simulink model "sf_aircraft"  (R2025b)
settings: configuration reference "SharedConfig" (kept outside this file)
PreLoadFcn:
  | load_system('sf_aircraft_lib.slx');
  | load_system('sf_aircraft_controller.slx');
model workspace (MAT data in the model file):
  reset_cmd = 0
values from neighbouring files (symbols this model uses):
  ActuatorModeType : value not decoded    [sf_aircraft_dd.sldd]
undefined symbols (not defined in the file or in its folder): Left, noise_factor, Right
libraries: simulink x15, sf_aircraft_lib x4, SignalEditorBlockLib x1
(part 1 of 2)
settings Model: DataDictionary=sf_aircraft_dd.sldd  PacingRate=2  VariantFading=off  Creator=The MathWorks, Inc.  LastModifiedBy=The MathWorks, Inc.
settings ConfigSetRef: SourceName=SharedConfig

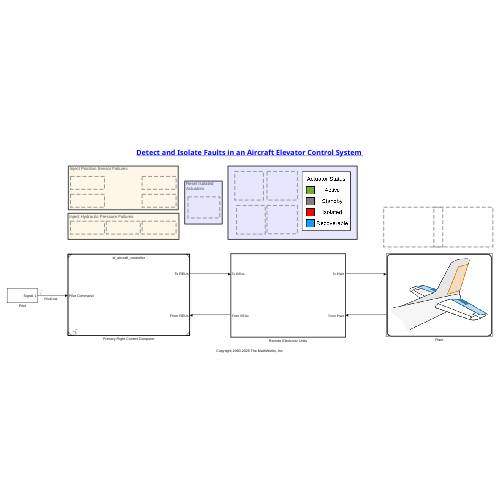
[thumbnail: Simulink's stored preview of the top-level diagram]
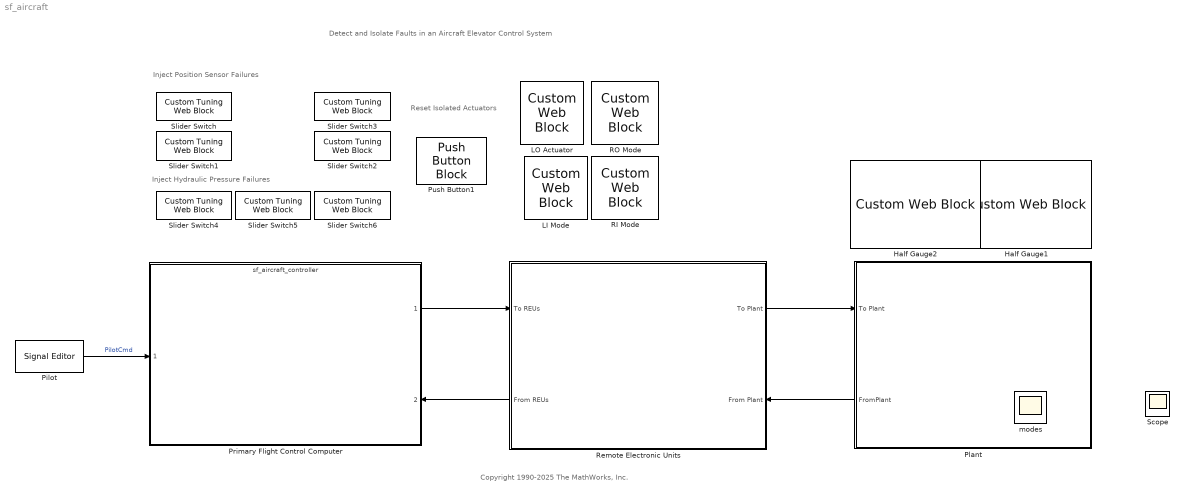
== system sf_aircraft ==
  note: Reset Isolated
      | Actuators
  note: Inject Hydraulic Pressure Failures
  note: Inject Position Sensor Failures
  note: Copyright 1990-2025 The MathWorks, Inc.
  note: Detect and Isolate Faults in an Aircraft Elevator Control System
  Half Gauge1 : CustomWebBlock  LabelPosition=Bottom  ShowInitialText=on  Configuration="{\"components\":[{\"name\":\"CircularScaleComponent\",\"settings\":{\"bounds\":{\"max\":1,\"min\":-1,\"tickInterval\":\"auto\"},\"direction\":\"cw\",\"flipLimits\":0,\"innerRadius\":0.75,\"internalTickHeightScaleFactor\":1,\"labelColor\":[255,255,200],\"labelFont\":{\"font\":\"Arial\",\"fontSize\":12},\"labelRadius\":0.528,\"labelTransparency\":1,\"minorTickHeightScaleFactor\":0.2,\"needleImage\":{\"size\":[200,50],\"src\":\"data:image\\/svg+xml;base64,PD94bWwgdmVyc2lvbj0iMS4wIiBlbmNvZGluZz0idXRmLTgiPz4KPCEtLSBHZW5lcmF0b3I6IEFkb2JlIElsbHVzdHJhdG9yIDI0LjEuMiwgU1ZHIEV4cG9ydCBQbHVnLUluIC4gU1ZHIFZlcnNpb246IDYuMDAgQnVpbGQgMCkgIC0tPgo8c3ZnIHZlcnNpb249IjEuMSIgaWQ9IkxheWVyXzEiIHhtbG5zPSJodHRwOi8vd3d3LnczLm9yZy8yMDAwL3N2ZyIgeG1sbnM6eGxpbms9Imh0dHA6Ly93d3cudzMub3JnLzE5OTkveGxpbmsiIHg9IjBweCIgeT0iMHB4IgoJIHZpZXdCb3g9IjAgMCAyMDAgNTAiIHN0eWxlPSJlbmFibGUtYmFja2dyb3VuZDpuZXcgMCAwIDIwMCA1MDsiIHhtbDpzcGFjZT0icHJlc2VydmUiPgo8c3R5bGUgdHlwZT0idGV4dC9jc3MiPgoJLnN0MHtmaWxsOiNFQzIxMjc7fQo8L3N0eWxlPgo8cGF0aCBjbGFzcz0ic3QwIiBkPSJNMTYyLjgsMTMuN0MxNjksNC40LDE4MS43LDEuOSwxOTEsOC4xczExLjgsMTguOSw1LjYsMjguMnMtMTguOSwxMS44LTI4LjIsNS42bDAsMAoJQzE1OS4xLDM1LjYsMTU2LjYsMjMsMTYyLjgsMTMuN0wxNjIuOCwxMy43eiBNMTY1LjgsMTUuOGMtNS4xLDcuNi0zLjEsMTcuOSw0LjYsMjNjNy42LDUuMSwxNy45LDMuMSwyMy00LjYKCWM1LjEtNy42LDMuMS0xNy45LTQuNi0yM2wwLDBDMTgxLjIsNi4yLDE3MC45LDguMiwxNjUuOCwxNS44eiIvPgo8cGF0aCBjbGFzcz0ic3QwIiBkPSJNMC40LDI1Ljl2LTMuM2wxNTktMi41Yy0wLjcsMi42LTAuNyw1LjIsMCw3LjhMMC40LDI1Ljl6Ii8+CjxjaXJjbGUgY2xhc3M9InN0MCIgY3g9IjE3OS42IiBjeT0iMjQiIHI9IjAuNyIvPgo8L3N2Zz4K\"},\"needleOffset\":[0.18464878250906522,0],\"needleOrientation\":-45,\"needleRotation\":180,\"needleSize\":{\"height\":0.11741692305346914,\"width\":0.46108337545091255},\"outerRadius\":0.9,\"position\":[-0.030336850649350648,0.09429505813953488,0.6517684108527132,1.0800527597402598],\"referencePoint\":\"auto\",\"scaleAngle\":120,\"scaleAngleOffset\":300,\"scaleColors\":[],\"scaleColorsSize\":0.2,\"scaleDirection\":\"CCW\",\"scalePosition\":[0,0,1,1],\"showLabels\":1,\"showMinorTicks\":1,\"showSpanLine\":1,\"showTicks\":1,\"tickColor\":[252,252,197],\"tickTransparency\":1,\"valueBarColor\":[0,0,0],\"valueBarPosition\":[0,0,1,1],\"valueBarSize\":0.2,\"valueBarTransparency\":1}},{\"name\":\"BackgroundImageComponent\",\"settings\":{\"image\":{\"size\":[0,0],\"src\":\"default\",\"srcOrientation\":\"Right\"},\"position\":[0,0,1,1],\"scaleMode\":\"0\"}},{\"name\":\"ForegroundImageComponent\",\"settings\":{\"image\":{\"size\":[0,0],\"src\":\"default\",\"srcOrientation\":[]},\"isForeground\":1,\"position\":[0,0,1,1],\"scaleMode\":\"0\"}}],\"derived\":{\"blockParameters\":{\"ForegroundColor\":[0.9882352941176471,0.9882352941176471,0.7725490196078432],\"Limits\":{\"Max\":1,\"Min\":-1,\"Ticks\":\"auto\"},\"ScaleColors\":[],\"ScaleDirection\":\"Counterclockwise\",\"ScaleMax\":1,\"ScaleMin\":-1,\"TickInterval\":\"auto\",\"fixedAspectRatio\":\"off\"}},\"settings\":{\"BindingType\":\"signal\",\"aspectRatio\":1.032258064516129,\"backgroundColor\":[0,0,0,\"1\"],\"backgroundOffset\":1,\"backgroundOpacity\":1,\"direction\":\"cw\",\"fixedAspectRatio\":\"off\",\"flipLimits\":0,\"orientation\":\"horizontal\",\"showBackgroundColor\":false,\"value\":0,\"version\":\"R2023a\"},\"type\":\"CircularGauge\"}"  CustomBackgroundColor="{\"color\":[0,0,0],\"show\":true}"
  Half Gauge2 : CustomWebBlock  LabelPosition=Bottom  ShowInitialText=on  Configuration="{\"components\":[{\"name\":\"CircularScaleComponent\",\"settings\":{\"bounds\":{\"max\":1,\"min\":-1,\"tickInterval\":\"auto\"},\"direction\":\"cw\",\"flipLimits\":0,\"innerRadius\":0.75,\"internalTickHeightScaleFactor\":1,\"labelColor\":[255,255,200],\"labelFont\":{\"font\":\"Arial\",\"fontSize\":12},\"labelRadius\":0.528,\"labelTransparency\":1,\"minorTickHeightScaleFactor\":0.2,\"needleImage\":{\"size\":[200,50],\"src\":\"data:image\\/svg+xml;base64,PD94bWwgdmVyc2lvbj0iMS4wIiBlbmNvZGluZz0idXRmLTgiPz4KPCEtLSBHZW5lcmF0b3I6IEFkb2JlIElsbHVzdHJhdG9yIDI0LjEuMiwgU1ZHIEV4cG9ydCBQbHVnLUluIC4gU1ZHIFZlcnNpb246IDYuMDAgQnVpbGQgMCkgIC0tPgo8c3ZnIHZlcnNpb249IjEuMSIgaWQ9IkxheWVyXzEiIHhtbG5zPSJodHRwOi8vd3d3LnczLm9yZy8yMDAwL3N2ZyIgeG1sbnM6eGxpbms9Imh0dHA6Ly93d3cudzMub3JnLzE5OTkveGxpbmsiIHg9IjBweCIgeT0iMHB4IgoJIHZpZXdCb3g9IjAgMCAyMDAgNTAiIHN0eWxlPSJlbmFibGUtYmFja2dyb3VuZDpuZXcgMCAwIDIwMCA1MDsiIHhtbDpzcGFjZT0icHJlc2VydmUiPgo8c3R5bGUgdHlwZT0idGV4dC9jc3MiPgoJLnN0MHtmaWxsOiNFQzIxMjc7fQo8L3N0eWxlPgo8cGF0aCBjbGFzcz0ic3QwIiBkPSJNMTYyLjgsMTMuN0MxNjksNC40LDE4MS43LDEuOSwxOTEsOC4xczExLjgsMTguOSw1LjYsMjguMnMtMTguOSwxMS44LTI4LjIsNS42bDAsMAoJQzE1OS4xLDM1LjYsMTU2LjYsMjMsMTYyLjgsMTMuN0wxNjIuOCwxMy43eiBNMTY1LjgsMTUuOGMtNS4xLDcuNi0zLjEsMTcuOSw0LjYsMjNjNy42LDUuMSwxNy45LDMuMSwyMy00LjYKCWM1LjEtNy42LDMuMS0xNy45LTQuNi0yM2wwLDBDMTgxLjIsNi4yLDE3MC45LDguMiwxNjUuOCwxNS44eiIvPgo8cGF0aCBjbGFzcz0ic3QwIiBkPSJNMC40LDI1Ljl2LTMuM2wxNTktMi41Yy0wLjcsMi42LTAuNyw1LjIsMCw3LjhMMC40LDI1Ljl6Ii8+CjxjaXJjbGUgY2xhc3M9InN0MCIgY3g9IjE3OS42IiBjeT0iMjQiIHI9IjAuNyIvPgo8L3N2Zz4K\"},\"needleOffset\":[0.18464878250906522,0],\"needleOrientation\":-45,\"needleRotation\":180,\"needleSize\":{\"height\":0.11741692305346914,\"width\":0.46108337545091255},\"outerRadius\":0.9,\"position\":[-0.012416294642857142,0.28617619493908153,0.6517806935332708,1.080078125],\"referencePoint\":\"auto\",\"scaleAngle\":120,\"scaleAngleOffset\":120,\"scaleColors\":[],\"scaleColorsSize\":0.2,\"scaleDirection\":\"CW\",\"scalePosition\":[0,0,1,1],\"showLabels\":1,\"showMinorTicks\":1,\"showSpanLine\":1,\"showTicks\":1,\"tickColor\":[252,252,197],\"tickTransparency\":1,\"valueBarColor\":[0,0,0],\"valueBarPosition\":[0,0,1,1],\"valueBarSize\":0.2,\"valueBarTransparency\":1}},{\"name\":\"BackgroundImageComponent\",\"settings\":{\"image\":{\"size\":[0,0],\"src\":\"default\",\"srcOrientation\":\"Right\"},\"position\":[0,0,1,1],\"scaleMode\":\"0\"}},{\"name\":\"ForegroundImageComponent\",\"settings\":{\"image\":{\"size\":[0,0],\"src\":\"default\",\"srcOrientation\":[]},\"isForeground\":1,\"position\":[0,0,1,1],\"scaleMode\":\"0\"}}],\"derived\":{\"blockParameters\":{\"ForegroundColor\":[0.9882352941176471,0.9882352941176471,0.7725490196078432],\"Limits\":{\"Max\":1,\"Min\":-1,\"Ticks\":\"auto\"},\"ScaleColors\":[],\"ScaleDirection\":\"Clockwise\",\"ScaleMax\":1,\"ScaleMin\":-1,\"TickInterval\":\"auto\",\"fixedAspectRatio\":\"on\"}},\"settings\":{\"BindingType\":\"signal\",\"aspectRatio\":1.032258064516129,\"backgroundColor\":[0,0,0,\"1\"],\"backgroundOffset\":1,\"backgroundOpacity\":1,\"direction\":\"cw\",\"fixedAspectRatio\":\"on\",\"flipLimits\":0,\"orientation\":\"horizontal\",\"showBackgroundColor\":false,\"value\":0,\"version\":\"R2023a\"},\"type\":\"CircularGauge\"}"  CustomBackgroundColor="{\"color\":[0,0,0],\"show\":true}"
  LI Mode : CustomWebBlock  LabelPosition=Bottom  ShowInitialText=on  Configuration="{\"components\":[{\"name\":\"BackgroundImageComponent\",\"settings\":{\"image\":{\"size\":[150,150],\"src\":\"data:image\\/svg+xml;base64,PHN2ZyB4bWxucz0iaHR0cDovL3d3dy53My5vcmcvMjAwMC9zdmciIHhtbG5zOnhsaW5rPSJodHRwOi8vd3d3LnczLm9yZy8xOTk5L3hsaW5rIiB2aWV3Qm94PSIwIDAgNTAwIDUwMCI+PGRlZnM+PHN0eWxlPi5he2ZpbGw6dXJsKCNhKTt9LmJ7ZmlsbDp1cmwoI2IpO30uY3tmaWxsOnVybCgjYyk7fTwvc3R5bGU+PHJhZGlhbEdyYWRpZW50IGlkPSJhIiBjeD0iMjgzLjg0IiBjeT0iLTQ2Ni4zNyIgcj0iMzc1Ljc1IiBncmFkaWVudFRyYW5zZm9ybT0ibWF0cml4KDEuMzksIDAsIDAsIC0xLjM5LCAtMTUzLjU2LCAtNjQ0LjA4KSIg ...(+2088 chars)\",\"srcOrientation\":\"Right\"},\"position\":[0,0,1,1],\"scaleMode\":\"0\"}},{\"name\":\"LampStateComponent\",\"settings\":{\"position\":[0,0,1,1],\"states\":[{\"icon\":{\"customSrc\":\"data:image\\/svg+xml;base64,PHN2ZyBpZD0iTGF5ZXJfMSIgZGF0YS1uYW1lPSJMYXllciAxIiB4bWxucz0iaHR0cDovL3d3dy53My5vcmcvMjAwMC9zdmciIHZpZXdCb3g9IjAgMCA0MTEgNDU4Ij48ZGVmcz48c3R5bGU+LmNscy0xe2ZpbGw6I2ZkZjhjMTt9LmNscy0ye2ZpbGw6I2ZlZTEwMDt9LmNscy0ze2ZpbGw6IzIzMWYyMDt9LmNscy00e2ZpbGw6I2EwOWY5Zjt9LmNscy00LC5jbHMtNSwuY2xzLTZ7c3Ryb2tlOiMyMzFmMjA7c3Ryb2tlLW1pdGVybGltaXQ6MTA7fS5jbHMtNXtmaWxsOiNmZmY7fS5jbHMtNntmaWxsOm5vbmU7fTwvc3R5bGU+PC9kZWZz ...(+5168 chars)\",\"id\":-1,\"srcOrientation\":\"Right\",\"type\":\"custom\"},\"iconScale\":0.8,\"metadata\":{},\"overlayType\":\"intersect\",\"shape\":{\"color\":[0.725,0,0],\"opacity\":1,\"position\":[0.1,0.1,0.8,0.8],\"type\":\"ellipse\"},\"value\":[]},{\"icon\":{\"customSrc\":\"data:image\\/svg+xml;base64,PHN2ZyBpZD0iTGF5ZXJfMSIgZGF0YS1uYW1lPSJMYXllciAxIiB4bWxucz0iaHR0cDovL3d3dy53My5vcmcvMjAwMC9zdmciIHZpZXdCb3g9IjAgMCA0MTEgNDU4Ij48ZGVmcz48c3R5bGU+LmNscy0xe2ZpbGw6I2ZkZjhjMTt9LmNscy0ye2ZpbGw6I2ZlZTEwMDt9LmNscy0ze2ZpbGw6IzIzMWYyMDt9LmNscy00e2ZpbGw6I2EwOWY5Zjt9LmNscy00LC5jbHMtNSwuY2xzLTZ7c3Ryb2tlOiMyMzFmMjA7c3Ryb2tlLW1pdGVybGltaXQ6MTA7fS5jbHMtNXtmaWxsOiNmZmY7fS5jbHMtNntmaWxsOm5vbmU7fTwvc3R5bGU+PC9kZWZz ...(+5168 chars)\",\"id\":-1,\"srcOrientation\":\"Right\",\"type\":\"custom\"},\"iconScale\":0.8,\"metadata\":{\"useDefaults\":{\"customIcon\":true,\"icon\":true,\"overlayType\":true,\"shape\":true,\"sizeAndPosition\":true}},\"overlayType\":\"intersect\",\"shape\":{\"color\":[0,0,0],\"opacity\":1,\"position\":[0.1,0.1,0.8,0.8],\"type\":\"ellipse\"},\"value\":\"0\"},{\"icon\":{\"customSrc\":\"data:image\\/svg+xml;base64,PHN2ZyBpZD0iTGF5ZXJfMSIgZGF0YS1uYW1lPSJMYXllciAxIiB4bWxucz0iaHR0cDovL3d3dy53My5vcmcvMjAwMC9zdmciIHZpZXdCb3g9IjAgMCA0MTEgNDU4Ij48ZGVmcz48c3R5bGU+LmNscy0xe2ZpbGw6I2ZkZjhjMTt9LmNscy0ye2ZpbGw6I2ZlZTEwMDt9LmNscy0ze2ZpbGw6IzIzMWYyMDt9LmNscy00e2ZpbGw6I2EwOWY5Zjt9LmNscy00LC5jbHMtNSwuY2xzLTZ7c3Ryb2tlOiMyMzFmMjA7c3Ryb2tlLW1pdGVybGltaXQ6MTA7fS5jbHMtNXtmaWxsOiNmZmY7fS5jbHMtNntmaWxsOm5vbmU7fTwvc3R5bGU+PC9kZWZz ...(+5168 chars)\",\"id\":-1,\"srcOrientation\":\"Right\",\"type\":\"custom\"},\"iconScale\":0.8,\"metadata\":{\"useDefaults\":{\"customIcon\":true,\"icon\":true,\"overlayType\":true,\"shape\":true,\"sizeAndPosition\":true}},\"overlayType\":\"intersect\",\"shape\":{\"color\":[0.4666666666666667,0.6745098039215687,0.18823529411764706],\"opacity\":1,\"position\":[0.1,0.1,0.8,0.8],\"type\":\"ellipse\"},\"value\":\"1\"},{\"icon\":{\"customSrc\":\"data:image\\/svg+xml;base64,PHN2ZyBpZD0iTGF5ZXJfMSIgZGF0YS1uYW1lPSJMYXllciAxIiB4bWxucz0iaHR0cDovL3d3dy53My5vcmcvMjAwMC9zdmciIHZpZXdCb3g9IjAgMCA0MTEgNDU4Ij48ZGVmcz48c3R5bGU+LmNscy0xe2ZpbGw6I2ZkZjhjMTt9LmNscy0ye2ZpbGw6I2ZlZTEwMDt9LmNscy0ze2ZpbGw6IzIzMWYyMDt9LmNscy00e2ZpbGw6I2EwOWY5Zjt9LmNscy00LC5jbHMtNSwuY2xzLTZ7c3Ryb2tlOiMyMzFmMjA7c3Ryb2tlLW1pdGVybGltaXQ6MTA7fS5jbHMtNXtmaWxsOiNmZmY7fS5jbHMtNntmaWxsOm5vbmU7fTwvc3R5bGU+PC9kZWZz ...(+5168 chars)\",\"id\":-1,\"srcOrientation\":\"Right\",\"type\":\"custom\"},\"iconScale\":0.8,\"metadata\":{\"useDefaults\":{\"customIcon\":true,\"icon\":true,\"overlayType\":true,\"shape\":true,\"sizeAndPosition\":true}},\"overlayType\":\"intersect\",\"shape\":{\"color\":[0.5019607843137255,0.5019607843137255,0.5019607843137255],\"opacity\":1,\"position\":[0.1,0.1,0.8,0.8],\"type\":\"ellipse\"},\"value\":\"2\"},{\"icon\":{\"customSrc\":\"data:image\\/svg+xml;base64,PHN2ZyBpZD0iTGF5ZXJfMSIgZGF0YS1uYW1lPSJMYXllciAxIiB4bWxucz0iaHR0cDovL3d3dy53My5vcmcvMjAwMC9zdmciIHZpZXdCb3g9IjAgMCA0MTEgNDU4Ij48ZGVmcz48c3R5bGU+LmNscy0xe2ZpbGw6I2ZkZjhjMTt9LmNscy0ye2ZpbGw6I2ZlZTEwMDt9LmNscy0ze2ZpbGw6IzIzMWYyMDt9LmNscy00e2ZpbGw6I2EwOWY5Zjt9LmNscy00LC5jbHMtNSwuY2xzLTZ7c3Ryb2tlOiMyMzFmMjA7c3Ryb2tlLW1pdGVybGltaXQ6MTA7fS5jbHMtNXtmaWxsOiNmZmY7fS5jbHMtNntmaWxsOm5vbmU7fTwvc3R5bGU+PC9kZWZz ...(+5168 chars)\",\"id\":-1,\"srcOrientation\":\"Right\",\"type\":\"custom\"},\"iconScale\":0.8,\"metadata\":{\"useDefaults\":{\"customIcon\":true,\"icon\":true,\"overlayType\":true,\"shape\":true,\"sizeAndPosition\":true}},\"overlayType\":\"intersect\",\"shape\":{\"color\":[1,0,0],\"opacity\":1,\"position\":[0.1,0.1,0.8,0.8],\"type\":\"ellipse\"},\"value\":\"3\"},{\"icon\":{\"customSrc\":\"data:image\\/svg+xml;base64,PHN2ZyBpZD0iTGF5ZXJfMSIgZGF0YS1uYW1lPSJMYXllciAxIiB4bWxucz0iaHR0cDovL3d3dy53My5vcmcvMjAwMC9zdmciIHZpZXdCb3g9IjAgMCA0MTEgNDU4Ij48ZGVmcz48c3R5bGU+LmNscy0xe2ZpbGw6I2ZkZjhjMTt9LmNscy0ye2ZpbGw6I2ZlZTEwMDt9LmNscy0ze2ZpbGw6IzIzMWYyMDt9LmNscy00e2ZpbGw6I2EwOWY5Zjt9LmNscy00LC5jbHMtNSwuY2xzLTZ7c3Ryb2tlOiMyMzFmMjA7c3Ryb2tlLW1pdGVybGltaXQ6MTA7fS5jbHMtNXtmaWxsOiNmZmY7fS5jbHMtNntmaWxsOm5vbmU7fTwvc3R5bGU+PC9kZWZz ...(+5168 chars)\",\"id\":-1,\"srcOrientation\":\"Right\",\"type\":\"custom\"},\"iconScale\":0.8,\"metadata\":{\"useDefaults\":{\"customIcon\":true,\"icon\":true,\"overlayType\":true,\"shape\":true,\"sizeAndPosition\":true}},\"overlayType\":\"intersect\",\"shape\":{\"color\":[0.07450980392156863,0.6235294117647059,1],\"opacity\":1,\"position\":[0.1,0.1,0.8,0.8],\"type\":\"ellipse\"},\"value\":\"4\"}],\"valueType\":\"discrete\"}},{\"name\":\"ForegroundImageComponent\",\"settings\":{\"image\":{\"size\":[150,150],\"src\":\"data:image\\/svg+xml;base64,PHN2ZyB4bWxucz0iaHR0cDovL3d3dy53My5vcmcvMjAwMC9zdmciIHhtbG5zOnhsaW5rPSJodHRwOi8vd3d3LnczLm9yZy8xOTk5L3hsaW5rIiB2aWV3Qm94PSIwIDAgNTAwIDUwMCI+PGRlZnM+PHN0eWxlPi5he2ZpbGw6dXJsKCNhKTt9PC9zdHlsZT48bGluZWFyR3JhZGllbnQgaWQ9ImEiIHgxPSIxNzMuMDUiIHkxPSItNjI3Ljc4IiB4Mj0iMTczLjA1IiB5Mj0iLTUyMi40MyIgZ3JhZGllbnRUcmFuc2Zvcm09Im1hdHJpeCgxLjI5LCAwLCAwLCAtMS4zMywgMjcuMTMsIC02MjguMzEpIiBncmFkaWVudFVuaXRzPSJ1c2VyU3BhY2VPblVzZSI+PHN0b3Agb2Zmc2V0PSIwIiBzdG9wLWNvbG9yPSIjZmZmIiBzdG9wLW9wYWNpdHk9IjAuMjUiLz48c3RvcCBvZmZzZXQ9IjEiIHN0b3AtY29sb3I9IiNmZmYiIHN0b3Atb3BhY2l0eT0iMCIvPjwvbGluZWFyR3JhZGllbnQ+PC9kZWZzPjxwYXRoIGNsYXNzPSJhIiBkPSJNNDI5LjMsMTkwLjY2QzQwMi40NSwxMTQuNTEsMzMyLjY3LDYwLjE3LDI1MC44NSw2MC4xN2MtODMuNDMsMC0xNTQuMjgsNTYuNDItMTc5Ljk1LDEzNSwxNS4zNCwzOSw4OC4xMSw3LDE3Ny4wNyw3QzM0MCwyMDIuMDgsNDE3LjI2LDIzNi40Niw0MjkuMywxOTAuNjZaIi8+PC9zdmc+\",\"srcOrientation\":\"Right\"},\"isForeground\":1,\"position\":[0,0,1,1],\"scaleMode\":\"0\"}}],\"derived\":{\"blockParameters\":{\"CustomIcon\":\"data:image\\/svg+xml;base64,PHN2ZyBpZD0iTGF5ZXJfMSIgZGF0YS1uYW1lPSJMYXllciAxIiB4bWxucz0iaHR0cDovL3d3dy53My5vcmcvMjAwMC9zdmciIHZpZXdCb3g9IjAgMCA0MTEgNDU4Ij48ZGVmcz48c3R5bGU+LmNscy0xe2ZpbGw6I2ZkZjhjMTt9LmNscy0ye2ZpbGw6I2ZlZTEwMDt9LmNscy0ze2ZpbGw6IzIzMWYyMDt9LmNscy00e2ZpbGw6I2EwOWY5Zjt9LmNscy00LC5jbHMtNSwuY2xzLTZ7c3Ryb2tlOiMyMzFmMjA7c3Ryb2tlLW1pdGVybGltaXQ6MTA7fS5jbHMtNXtmaWxsOiNmZmY7fS5jbHMtNntmaWxsOm5vbmU7fTwvc3R5bGU+PC9kZWZz ...(+5168 chars)\",\"DefaultColor\":[0.725,0,0],\"Icon\":\"Custom\",\"StateColors\":[{\"color\":[0,0,0],\"value\":\"0\"},{\"color\":[0.4666666666666667,0.6745098039215687,0.18823529411764706],\"value\":\"1\"},{\"color\":[0.5019607843137255,0.5019607843137255,0.5019607843137255],\"value\":\"2\"},{\"color\":[1,0,0],\"value\":\"3\"},{\"color\":[0.07450980392156863,0.6235294117647059,1],\"value\":\"4\"}],\"StateValueType\":\"discrete\",\"fixedAspectRatio\":\"off\"}},\"settings\":{\"BindingType\":\"signal\",\"aspectRatio\":1.032258064516129,\"backgroundColor\":[0,0,0],\"backgroundOffset\":0.14,\"backgroundOpacity\":1,\"blockOrientation\":\"Right\",\"fixedAspectRatio\":\"off\",\"showBackgroundColor\":false,\"value\":0,\"version\":\"R2023a\"},\"type\":\"Lamp\"}"
  "LO Actuator  " : CustomWebBlock  LabelPosition=Bottom  ShowInitialText=on  Configuration="{\"components\":[{\"name\":\"BackgroundImageComponent\",\"settings\":{\"image\":{\"size\":[150,150],\"src\":\"data:image\\/svg+xml;base64,PHN2ZyB4bWxucz0iaHR0cDovL3d3dy53My5vcmcvMjAwMC9zdmciIHhtbG5zOnhsaW5rPSJodHRwOi8vd3d3LnczLm9yZy8xOTk5L3hsaW5rIiB2aWV3Qm94PSIwIDAgNTAwIDUwMCI+PGRlZnM+PHN0eWxlPi5he2ZpbGw6dXJsKCNhKTt9LmJ7ZmlsbDp1cmwoI2IpO30uY3tmaWxsOnVybCgjYyk7fTwvc3R5bGU+PHJhZGlhbEdyYWRpZW50IGlkPSJhIiBjeD0iMjgzLjg0IiBjeT0iLTQ2Ni4zNyIgcj0iMzc1Ljc1IiBncmFkaWVudFRyYW5zZm9ybT0ibWF0cml4KDEuMzksIDAsIDAsIC0xLjM5LCAtMTUzLjU2LCAtNjQ0LjA4KSIg ...(+2088 chars)\",\"srcOrientation\":\"Right\"},\"position\":[0,0,1,1],\"scaleMode\":\"0\"}},{\"name\":\"LampStateComponent\",\"settings\":{\"position\":[0,0,1,1],\"states\":[{\"icon\":{\"customSrc\":\"data:image\\/svg+xml;base64,PHN2ZyBpZD0iTGF5ZXJfMSIgZGF0YS1uYW1lPSJMYXllciAxIiB4bWxucz0iaHR0cDovL3d3dy53My5vcmcvMjAwMC9zdmciIHZpZXdCb3g9IjAgMCA0MTEgNDU4Ij48ZGVmcz48c3R5bGU+LmNscy0xe2ZpbGw6I2ZkZjhjMTt9LmNscy0ye2ZpbGw6I2ZlZTEwMDt9LmNscy0ze2ZpbGw6IzIzMWYyMDt9LmNscy00e2ZpbGw6I2EwOWY5Zjt9LmNscy00LC5jbHMtNSwuY2xzLTZ7c3Ryb2tlOiMyMzFmMjA7c3Ryb2tlLW1pdGVybGltaXQ6MTA7fS5jbHMtNXtmaWxsOiNmZmY7fS5jbHMtNntmaWxsOm5vbmU7fTwvc3R5bGU+PC9kZWZz ...(+5168 chars)\",\"id\":-1,\"srcOrientation\":\"Right\",\"type\":\"custom\"},\"iconScale\":0.8,\"metadata\":{},\"overlayType\":\"intersect\",\"shape\":{\"color\":[0.725,0,0],\"opacity\":1,\"position\":[0.1,0.1,0.8,0.8],\"type\":\"ellipse\"},\"value\":[]},{\"icon\":{\"customSrc\":\"data:image\\/svg+xml;base64,PHN2ZyBpZD0iTGF5ZXJfMSIgZGF0YS1uYW1lPSJMYXllciAxIiB4bWxucz0iaHR0cDovL3d3dy53My5vcmcvMjAwMC9zdmciIHZpZXdCb3g9IjAgMCA0MTEgNDU4Ij48ZGVmcz48c3R5bGU+LmNscy0xe2ZpbGw6I2ZkZjhjMTt9LmNscy0ye2ZpbGw6I2ZlZTEwMDt9LmNscy0ze2ZpbGw6IzIzMWYyMDt9LmNscy00e2ZpbGw6I2EwOWY5Zjt9LmNscy00LC5jbHMtNSwuY2xzLTZ7c3Ryb2tlOiMyMzFmMjA7c3Ryb2tlLW1pdGVybGltaXQ6MTA7fS5jbHMtNXtmaWxsOiNmZmY7fS5jbHMtNntmaWxsOm5vbmU7fTwvc3R5bGU+PC9kZWZz ...(+5168 chars)\",\"id\":-1,\"srcOrientation\":\"Right\",\"type\":\"custom\"},\"iconScale\":0.8,\"metadata\":{\"useDefaults\":{\"customIcon\":true,\"icon\":true,\"overlayType\":true,\"shape\":true,\"sizeAndPosition\":true}},\"overlayType\":\"intersect\",\"shape\":{\"color\":[0,0,0],\"opacity\":1,\"position\":[0.1,0.1,0.8,0.8],\"type\":\"ellipse\"},\"value\":\"0\"},{\"icon\":{\"customSrc\":\"data:image\\/svg+xml;base64,PHN2ZyBpZD0iTGF5ZXJfMSIgZGF0YS1uYW1lPSJMYXllciAxIiB4bWxucz0iaHR0cDovL3d3dy53My5vcmcvMjAwMC9zdmciIHZpZXdCb3g9IjAgMCA0MTEgNDU4Ij48ZGVmcz48c3R5bGU+LmNscy0xe2ZpbGw6I2ZkZjhjMTt9LmNscy0ye2ZpbGw6I2ZlZTEwMDt9LmNscy0ze2ZpbGw6IzIzMWYyMDt9LmNscy00e2ZpbGw6I2EwOWY5Zjt9LmNscy00LC5jbHMtNSwuY2xzLTZ7c3Ryb2tlOiMyMzFmMjA7c3Ryb2tlLW1pdGVybGltaXQ6MTA7fS5jbHMtNXtmaWxsOiNmZmY7fS5jbHMtNntmaWxsOm5vbmU7fTwvc3R5bGU+PC9kZWZz ...(+5168 chars)\",\"id\":-1,\"srcOrientation\":\"Right\",\"type\":\"custom\"},\"iconScale\":0.8,\"metadata\":{\"useDefaults\":{\"customIcon\":true,\"icon\":true,\"overlayType\":true,\"shape\":true,\"sizeAndPosition\":true}},\"overlayType\":\"intersect\",\"shape\":{\"color\":[0.4666666666666667,0.6745098039215687,0.18823529411764706],\"opacity\":1,\"position\":[0.1,0.1,0.8,0.8],\"type\":\"ellipse\"},\"value\":\"1\"},{\"icon\":{\"customSrc\":\"data:image\\/svg+xml;base64,PHN2ZyBpZD0iTGF5ZXJfMSIgZGF0YS1uYW1lPSJMYXllciAxIiB4bWxucz0iaHR0cDovL3d3dy53My5vcmcvMjAwMC9zdmciIHZpZXdCb3g9IjAgMCA0MTEgNDU4Ij48ZGVmcz48c3R5bGU+LmNscy0xe2ZpbGw6I2ZkZjhjMTt9LmNscy0ye2ZpbGw6I2ZlZTEwMDt9LmNscy0ze2ZpbGw6IzIzMWYyMDt9LmNscy00e2ZpbGw6I2EwOWY5Zjt9LmNscy00LC5jbHMtNSwuY2xzLTZ7c3Ryb2tlOiMyMzFmMjA7c3Ryb2tlLW1pdGVybGltaXQ6MTA7fS5jbHMtNXtmaWxsOiNmZmY7fS5jbHMtNntmaWxsOm5vbmU7fTwvc3R5bGU+PC9kZWZz ...(+5168 chars)\",\"id\":-1,\"srcOrientation\":\"Right\",\"type\":\"custom\"},\"iconScale\":0.8,\"metadata\":{\"useDefaults\":{\"customIcon\":true,\"icon\":true,\"overlayType\":true,\"shape\":true,\"sizeAndPosition\":true}},\"overlayType\":\"intersect\",\"shape\":{\"color\":[0.5019607843137255,0.5019607843137255,0.5019607843137255],\"opacity\":1,\"position\":[0.1,0.1,0.8,0.8],\"type\":\"ellipse\"},\"value\":\"2\"},{\"icon\":{\"customSrc\":\"data:image\\/svg+xml;base64,PHN2ZyBpZD0iTGF5ZXJfMSIgZGF0YS1uYW1lPSJMYXllciAxIiB4bWxucz0iaHR0cDovL3d3dy53My5vcmcvMjAwMC9zdmciIHZpZXdCb3g9IjAgMCA0MTEgNDU4Ij48ZGVmcz48c3R5bGU+LmNscy0xe2ZpbGw6I2ZkZjhjMTt9LmNscy0ye2ZpbGw6I2ZlZTEwMDt9LmNscy0ze2ZpbGw6IzIzMWYyMDt9LmNscy00e2ZpbGw6I2EwOWY5Zjt9LmNscy00LC5jbHMtNSwuY2xzLTZ7c3Ryb2tlOiMyMzFmMjA7c3Ryb2tlLW1pdGVybGltaXQ6MTA7fS5jbHMtNXtmaWxsOiNmZmY7fS5jbHMtNntmaWxsOm5vbmU7fTwvc3R5bGU+PC9kZWZz ...(+5168 chars)\",\"id\":-1,\"srcOrientation\":\"Right\",\"type\":\"custom\"},\"iconScale\":0.8,\"metadata\":{\"useDefaults\":{\"customIcon\":true,\"icon\":true,\"overlayType\":true,\"shape\":true,\"sizeAndPosition\":true}},\"overlayType\":\"intersect\",\"shape\":{\"color\":[1,0,0],\"opacity\":1,\"position\":[0.1,0.1,0.8,0.8],\"type\":\"ellipse\"},\"value\":\"3\"},{\"icon\":{\"customSrc\":\"data:image\\/svg+xml;base64,PHN2ZyBpZD0iTGF5ZXJfMSIgZGF0YS1uYW1lPSJMYXllciAxIiB4bWxucz0iaHR0cDovL3d3dy53My5vcmcvMjAwMC9zdmciIHZpZXdCb3g9IjAgMCA0MTEgNDU4Ij48ZGVmcz48c3R5bGU+LmNscy0xe2ZpbGw6I2ZkZjhjMTt9LmNscy0ye2ZpbGw6I2ZlZTEwMDt9LmNscy0ze2ZpbGw6IzIzMWYyMDt9LmNscy00e2ZpbGw6I2EwOWY5Zjt9LmNscy00LC5jbHMtNSwuY2xzLTZ7c3Ryb2tlOiMyMzFmMjA7c3Ryb2tlLW1pdGVybGltaXQ6MTA7fS5jbHMtNXtmaWxsOiNmZmY7fS5jbHMtNntmaWxsOm5vbmU7fTwvc3R5bGU+PC9kZWZz ...(+5168 chars)\",\"id\":-1,\"srcOrientation\":\"Right\",\"type\":\"custom\"},\"iconScale\":0.8,\"metadata\":{\"useDefaults\":{\"customIcon\":true,\"icon\":true,\"overlayType\":true,\"shape\":true,\"sizeAndPosition\":true}},\"overlayType\":\"intersect\",\"shape\":{\"color\":[0.07450980392156863,0.6235294117647059,1],\"opacity\":1,\"position\":[0.1,0.1,0.8,0.8],\"type\":\"ellipse\"},\"value\":\"4\"}],\"valueType\":\"discrete\"}},{\"name\":\"ForegroundImageComponent\",\"settings\":{\"image\":{\"size\":[150,150],\"src\":\"data:image\\/svg+xml;base64,PHN2ZyB4bWxucz0iaHR0cDovL3d3dy53My5vcmcvMjAwMC9zdmciIHhtbG5zOnhsaW5rPSJodHRwOi8vd3d3LnczLm9yZy8xOTk5L3hsaW5rIiB2aWV3Qm94PSIwIDAgNTAwIDUwMCI+PGRlZnM+PHN0eWxlPi5he2ZpbGw6dXJsKCNhKTt9PC9zdHlsZT48bGluZWFyR3JhZGllbnQgaWQ9ImEiIHgxPSIxNzMuMDUiIHkxPSItNjI3Ljc4IiB4Mj0iMTczLjA1IiB5Mj0iLTUyMi40MyIgZ3JhZGllbnRUcmFuc2Zvcm09Im1hdHJpeCgxLjI5LCAwLCAwLCAtMS4zMywgMjcuMTMsIC02MjguMzEpIiBncmFkaWVudFVuaXRzPSJ1c2VyU3BhY2VPblVzZSI+PHN0b3Agb2Zmc2V0PSIwIiBzdG9wLWNvbG9yPSIjZmZmIiBzdG9wLW9wYWNpdHk9IjAuMjUiLz48c3RvcCBvZmZzZXQ9IjEiIHN0b3AtY29sb3I9IiNmZmYiIHN0b3Atb3BhY2l0eT0iMCIvPjwvbGluZWFyR3JhZGllbnQ+PC9kZWZzPjxwYXRoIGNsYXNzPSJhIiBkPSJNNDI5LjMsMTkwLjY2QzQwMi40NSwxMTQuNTEsMzMyLjY3LDYwLjE3LDI1MC44NSw2MC4xN2MtODMuNDMsMC0xNTQuMjgsNTYuNDItMTc5Ljk1LDEzNSwxNS4zNCwzOSw4OC4xMSw3LDE3Ny4wNyw3QzM0MCwyMDIuMDgsNDE3LjI2LDIzNi40Niw0MjkuMywxOTAuNjZaIi8+PC9zdmc+\",\"srcOrientation\":\"Right\"},\"isForeground\":1,\"position\":[0,0,1,1],\"scaleMode\":\"0\"}}],\"derived\":{\"blockParameters\":{\"CustomIcon\":\"data:image\\/svg+xml;base64,PHN2ZyBpZD0iTGF5ZXJfMSIgZGF0YS1uYW1lPSJMYXllciAxIiB4bWxucz0iaHR0cDovL3d3dy53My5vcmcvMjAwMC9zdmciIHZpZXdCb3g9IjAgMCA0MTEgNDU4Ij48ZGVmcz48c3R5bGU+LmNscy0xe2ZpbGw6I2ZkZjhjMTt9LmNscy0ye2ZpbGw6I2ZlZTEwMDt9LmNscy0ze2ZpbGw6IzIzMWYyMDt9LmNscy00e2ZpbGw6I2EwOWY5Zjt9LmNscy00LC5jbHMtNSwuY2xzLTZ7c3Ryb2tlOiMyMzFmMjA7c3Ryb2tlLW1pdGVybGltaXQ6MTA7fS5jbHMtNXtmaWxsOiNmZmY7fS5jbHMtNntmaWxsOm5vbmU7fTwvc3R5bGU+PC9kZWZz ...(+5168 chars)\",\"DefaultColor\":[0.725,0,0],\"Icon\":\"Custom\",\"StateColors\":[{\"color\":[0,0,0],\"value\":\"0\"},{\"color\":[0.4666666666666667,0.6745098039215687,0.18823529411764706],\"value\":\"1\"},{\"color\":[0.5019607843137255,0.5019607843137255,0.5019607843137255],\"value\":\"2\"},{\"color\":[1,0,0],\"value\":\"3\"},{\"color\":[0.07450980392156863,0.6235294117647059,1],\"value\":\"4\"}],\"StateValueType\":\"discrete\",\"fixedAspectRatio\":\"off\"}},\"settings\":{\"BindingType\":\"signal\",\"aspectRatio\":1.032258064516129,\"backgroundColor\":[0,0,0],\"backgroundOffset\":0.14,\"backgroundOpacity\":1,\"blockOrientation\":\"Right\",\"fixedAspectRatio\":\"off\",\"showBackgroundColor\":false,\"value\":0,\"version\":\"R2023a\"},\"type\":\"Lamp\"}"
  Pilot : SignalEditorBlockLib/Signal Editor  FileName=simplepilot.mat  ActiveScenario=Takeoff  ActiveSignal=Signal 1  IsBus=off  OutputBusObjectStr=Bus: BusObject  SampleTime=.1  Interpolate=off  ZeroCross=off  OutputAfterFinalValue=Setting to zero  Unit=inherit  PreserveSignalName=on  ApplySigPropsToAllScenarios=on  ApplySigPropsToAllSignals=off  SignalPropertySource=Dialog parameters
  Plant : Subsystem
      settings: PortSchema="{\"entries\":[{\"content\":{\"sides\":[{\"content\":{\"connectorIds\":[\"In1\",\"Out1\"]},\"type\":\"ConnectorPlacement.EquallySpacedRectSide\",\"uuid\":\"38682bff-efe9-4f74-b563-7d17327409bc\"},{\"content\":{\"side\":\"RIGHT\"},\"type\":\"ConnectorPlacement.EquallySpacedRectSide\",\"uuid\":\"9b27296a-7a15-43c2-9a49-3690713ba5ee\"},{\"content\":{\"side\":\"TOP\"},\"type\":\"ConnectorPlacement.EquallySpacedRectSide\",\"uuid\":\"df0d1eaf-2d63-4586-9b70-ab9eb3cbba48\"}]},\"type\":\"ConnectorPlacement.EquallySpacedConnector\",\"uuid\":\"3720bb81-e23a-4071-aa80-868b0be59702\"}],\"packageUris\":[\"http://schema.mathworks.com/mf0/Connector/R2020b\"],\"version\":\"1.0\"}"
      mask Display: image('aircraft-elevator.png');
  Primary Flight Control Computer : ModelReference  ModelNameDialog=sf_aircraft_controller  SimulationMode=Normal  ModelReferenceVersion=2.13
      settings: PortSchema="{\"entries\":[{\"content\":{\"sides\":[{\"content\":{\"connectorIds\":[\"In1\"]},\"type\":\"ConnectorPlacement.EquallySpacedRectSide\",\"uuid\":\"4aa03f90-93a0-4c7f-a3cd-6daab17b3951\"},{\"content\":{\"connectorIds\":[\"Out1\",\"In2\"],\"side\":\"RIGHT\"},\"type\":\"ConnectorPlacement.EquallySpacedRectSide\",\"uuid\":\"3b750c9f-37e0-4721-beac-0d825a86c64b\"},{\"content\":{\"side\":\"TOP\"},\"type\":\"ConnectorPlacement.EquallySpacedRectSide\",\"uuid\":\"845b3102-9354-404f-9f20-8ca6a930b73c\"}]},\"type\":\"ConnectorPlacement.EquallySpacedConnector\",\"uuid\":\"f07501ae-eb53-443d-bbea-7ab38e30640c\"}],\"packageUris\":[\"http://schema.mathworks.com/mf0/Connector/R2020b\"],\"version\":\"1.0\"}"
  Push Button1 : PushButtonBlock  Icon=Custom  CustomIcon=data:image/png;base64,iVBORw0KGgoAAAANSUhEUgAABQAAAAQyCAYAAAD3IVLlAAVlcklEQVR42uyYP2gUQRSHL/FSCNrYWIhgYSUIgmCZYKWFjUUqRXBnNrszk7vNxuSSS3ONFgpaiAiKXiGBoEK0sFAMiohCCsV/CCrEIoUBISQ7s94lJvf87XJwsTaN4X3wMe+9mTePZbotMAzDMAzDbEWoUOiq1WrdlNnfvy0TcZFqfcV7WUzUVdgknvfh3lFv54IQuxtBsC8pBQdSJQ8n2ut1oTyWGHnSKnE6NdI45Y84JaqJljUbyvNWy4tOySuJFtdSLW8gr2N/Et6F08gfwSfOiGfIX1olZ+Fb9HxE/sVqMYd13mm5gHgRscWsJnpacC2LocPeEnp+ovcH4nn4HfWv6PuMng+o ...(+471212 chars)  IconAlignment=Top  IconOnColor=[0.0, 0.39215686274509803, 0.0]  IconOffColor=[0.0, 1.0, 0.0]  OffValue=0.000000
  RI Mode : CustomWebBlock  LabelPosition=Bottom  ShowInitialText=on  Configuration="{\"components\":[{\"name\":\"BackgroundImageComponent\",\"settings\":{\"image\":{\"size\":[150,150],\"src\":\"data:image\\/svg+xml;base64,PHN2ZyB4bWxucz0iaHR0cDovL3d3dy53My5vcmcvMjAwMC9zdmciIHhtbG5zOnhsaW5rPSJodHRwOi8vd3d3LnczLm9yZy8xOTk5L3hsaW5rIiB2aWV3Qm94PSIwIDAgNTAwIDUwMCI+PGRlZnM+PHN0eWxlPi5he2ZpbGw6dXJsKCNhKTt9LmJ7ZmlsbDp1cmwoI2IpO30uY3tmaWxsOnVybCgjYyk7fTwvc3R5bGU+PHJhZGlhbEdyYWRpZW50IGlkPSJhIiBjeD0iMjgzLjg0IiBjeT0iLTQ2Ni4zNyIgcj0iMzc1Ljc1IiBncmFkaWVudFRyYW5zZm9ybT0ibWF0cml4KDEuMzksIDAsIDAsIC0xLjM5LCAtMTUzLjU2LCAtNjQ0LjA4KSIg ...(+2088 chars)\",\"srcOrientation\":\"Right\"},\"position\":[0,0,1,1],\"scaleMode\":\"0\"}},{\"name\":\"LampStateComponent\",\"settings\":{\"position\":[0,0,1,1],\"states\":[{\"icon\":{\"customSrc\":\"data:image\\/svg+xml;base64,PHN2ZyBpZD0iTGF5ZXJfMSIgZGF0YS1uYW1lPSJMYXllciAxIiB4bWxucz0iaHR0cDovL3d3dy53My5vcmcvMjAwMC9zdmciIHZpZXdCb3g9IjAgMCA0MTEgNDU4Ij48ZGVmcz48c3R5bGU+LmNscy0xe2ZpbGw6I2ZkZjhjMTt9LmNscy0ye2ZpbGw6I2ZlZTEwMDt9LmNscy0ze2ZpbGw6IzIzMWYyMDt9LmNscy00e2ZpbGw6I2EwOWY5Zjt9LmNscy00LC5jbHMtNSwuY2xzLTZ7c3Ryb2tlOiMyMzFmMjA7c3Ryb2tlLW1pdGVybGltaXQ6MTA7fS5jbHMtNXtmaWxsOiNmZmY7fS5jbHMtNntmaWxsOm5vbmU7fTwvc3R5bGU+PC9kZWZz ...(+5168 chars)\",\"id\":-1,\"srcOrientation\":\"Right\",\"type\":\"custom\"},\"iconScale\":0.8,\"metadata\":{},\"overlayType\":\"intersect\",\"shape\":{\"color\":[0.725,0,0],\"opacity\":1,\"position\":[0.1,0.1,0.8,0.8],\"type\":\"ellipse\"},\"value\":[]},{\"icon\":{\"customSrc\":\"data:image\\/svg+xml;base64,PHN2ZyBpZD0iTGF5ZXJfMSIgZGF0YS1uYW1lPSJMYXllciAxIiB4bWxucz0iaHR0cDovL3d3dy53My5vcmcvMjAwMC9zdmciIHZpZXdCb3g9IjAgMCA0MTEgNDU4Ij48ZGVmcz48c3R5bGU+LmNscy0xe2ZpbGw6I2ZkZjhjMTt9LmNscy0ye2ZpbGw6I2ZlZTEwMDt9LmNscy0ze2ZpbGw6IzIzMWYyMDt9LmNscy00e2ZpbGw6I2EwOWY5Zjt9LmNscy00LC5jbHMtNSwuY2xzLTZ7c3Ryb2tlOiMyMzFmMjA7c3Ryb2tlLW1pdGVybGltaXQ6MTA7fS5jbHMtNXtmaWxsOiNmZmY7fS5jbHMtNntmaWxsOm5vbmU7fTwvc3R5bGU+PC9kZWZz ...(+5168 chars)\",\"id\":-1,\"srcOrientation\":\"Right\",\"type\":\"custom\"},\"iconScale\":0.8,\"metadata\":{\"useDefaults\":{\"customIcon\":true,\"icon\":true,\"overlayType\":true,\"shape\":true,\"sizeAndPosition\":true}},\"overlayType\":\"intersect\",\"shape\":{\"color\":[0,0,0],\"opacity\":1,\"position\":[0.1,0.1,0.8,0.8],\"type\":\"ellipse\"},\"value\":\"0\"},{\"icon\":{\"customSrc\":\"data:image\\/svg+xml;base64,PHN2ZyBpZD0iTGF5ZXJfMSIgZGF0YS1uYW1lPSJMYXllciAxIiB4bWxucz0iaHR0cDovL3d3dy53My5vcmcvMjAwMC9zdmciIHZpZXdCb3g9IjAgMCA0MTEgNDU4Ij48ZGVmcz48c3R5bGU+LmNscy0xe2ZpbGw6I2ZkZjhjMTt9LmNscy0ye2ZpbGw6I2ZlZTEwMDt9LmNscy0ze2ZpbGw6IzIzMWYyMDt9LmNscy00e2ZpbGw6I2EwOWY5Zjt9LmNscy00LC5jbHMtNSwuY2xzLTZ7c3Ryb2tlOiMyMzFmMjA7c3Ryb2tlLW1pdGVybGltaXQ6MTA7fS5jbHMtNXtmaWxsOiNmZmY7fS5jbHMtNntmaWxsOm5vbmU7fTwvc3R5bGU+PC9kZWZz ...(+5168 chars)\",\"id\":-1,\"srcOrientation\":\"Right\",\"type\":\"custom\"},\"iconScale\":0.8,\"metadata\":{\"useDefaults\":{\"customIcon\":true,\"icon\":true,\"overlayType\":true,\"shape\":true,\"sizeAndPosition\":true}},\"overlayType\":\"intersect\",\"shape\":{\"color\":[0.4666666666666667,0.6745098039215687,0.18823529411764706],\"opacity\":1,\"position\":[0.1,0.1,0.8,0.8],\"type\":\"ellipse\"},\"value\":\"1\"},{\"icon\":{\"customSrc\":\"data:image\\/svg+xml;base64,PHN2ZyBpZD0iTGF5ZXJfMSIgZGF0YS1uYW1lPSJMYXllciAxIiB4bWxucz0iaHR0cDovL3d3dy53My5vcmcvMjAwMC9zdmciIHZpZXdCb3g9IjAgMCA0MTEgNDU4Ij48ZGVmcz48c3R5bGU+LmNscy0xe2ZpbGw6I2ZkZjhjMTt9LmNscy0ye2ZpbGw6I2ZlZTEwMDt9LmNscy0ze2ZpbGw6IzIzMWYyMDt9LmNscy00e2ZpbGw6I2EwOWY5Zjt9LmNscy00LC5jbHMtNSwuY2xzLTZ7c3Ryb2tlOiMyMzFmMjA7c3Ryb2tlLW1pdGVybGltaXQ6MTA7fS5jbHMtNXtmaWxsOiNmZmY7fS5jbHMtNntmaWxsOm5vbmU7fTwvc3R5bGU+PC9kZWZz ...(+5168 chars)\",\"id\":-1,\"srcOrientation\":\"Right\",\"type\":\"custom\"},\"iconScale\":0.8,\"metadata\":{\"useDefaults\":{\"customIcon\":true,\"icon\":true,\"overlayType\":true,\"shape\":true,\"sizeAndPosition\":true}},\"overlayType\":\"intersect\",\"shape\":{\"color\":[0.5019607843137255,0.5019607843137255,0.5019607843137255],\"opacity\":1,\"position\":[0.1,0.1,0.8,0.8],\"type\":\"ellipse\"},\"value\":\"2\"},{\"icon\":{\"customSrc\":\"data:image\\/svg+xml;base64,PHN2ZyBpZD0iTGF5ZXJfMSIgZGF0YS1uYW1lPSJMYXllciAxIiB4bWxucz0iaHR0cDovL3d3dy53My5vcmcvMjAwMC9zdmciIHZpZXdCb3g9IjAgMCA0MTEgNDU4Ij48ZGVmcz48c3R5bGU+LmNscy0xe2ZpbGw6I2ZkZjhjMTt9LmNscy0ye2ZpbGw6I2ZlZTEwMDt9LmNscy0ze2ZpbGw6IzIzMWYyMDt9LmNscy00e2ZpbGw6I2EwOWY5Zjt9LmNscy00LC5jbHMtNSwuY2xzLTZ7c3Ryb2tlOiMyMzFmMjA7c3Ryb2tlLW1pdGVybGltaXQ6MTA7fS5jbHMtNXtmaWxsOiNmZmY7fS5jbHMtNntmaWxsOm5vbmU7fTwvc3R5bGU+PC9kZWZz ...(+5168 chars)\",\"id\":-1,\"srcOrientation\":\"Right\",\"type\":\"custom\"},\"iconScale\":0.8,\"metadata\":{\"useDefaults\":{\"customIcon\":true,\"icon\":true,\"overlayType\":true,\"shape\":true,\"sizeAndPosition\":true}},\"overlayType\":\"intersect\",\"shape\":{\"color\":[1,0,0],\"opacity\":1,\"position\":[0.1,0.1,0.8,0.8],\"type\":\"ellipse\"},\"value\":\"3\"},{\"icon\":{\"customSrc\":\"data:image\\/svg+xml;base64,PHN2ZyBpZD0iTGF5ZXJfMSIgZGF0YS1uYW1lPSJMYXllciAxIiB4bWxucz0iaHR0cDovL3d3dy53My5vcmcvMjAwMC9zdmciIHZpZXdCb3g9IjAgMCA0MTEgNDU4Ij48ZGVmcz48c3R5bGU+LmNscy0xe2ZpbGw6I2ZkZjhjMTt9LmNscy0ye2ZpbGw6I2ZlZTEwMDt9LmNscy0ze2ZpbGw6IzIzMWYyMDt9LmNscy00e2ZpbGw6I2EwOWY5Zjt9LmNscy00LC5jbHMtNSwuY2xzLTZ7c3Ryb2tlOiMyMzFmMjA7c3Ryb2tlLW1pdGVybGltaXQ6MTA7fS5jbHMtNXtmaWxsOiNmZmY7fS5jbHMtNntmaWxsOm5vbmU7fTwvc3R5bGU+PC9kZWZz ...(+5168 chars)\",\"id\":-1,\"srcOrientation\":\"Right\",\"type\":\"custom\"},\"iconScale\":0.8,\"metadata\":{\"useDefaults\":{\"customIcon\":true,\"icon\":true,\"overlayType\":true,\"shape\":true,\"sizeAndPosition\":true}},\"overlayType\":\"intersect\",\"shape\":{\"color\":[0.07450980392156863,0.6235294117647059,1],\"opacity\":1,\"position\":[0.1,0.1,0.8,0.8],\"type\":\"ellipse\"},\"value\":\"4\"}],\"valueType\":\"discrete\"}},{\"name\":\"ForegroundImageComponent\",\"settings\":{\"image\":{\"size\":[150,150],\"src\":\"data:image\\/svg+xml;base64,PHN2ZyB4bWxucz0iaHR0cDovL3d3dy53My5vcmcvMjAwMC9zdmciIHhtbG5zOnhsaW5rPSJodHRwOi8vd3d3LnczLm9yZy8xOTk5L3hsaW5rIiB2aWV3Qm94PSIwIDAgNTAwIDUwMCI+PGRlZnM+PHN0eWxlPi5he2ZpbGw6dXJsKCNhKTt9PC9zdHlsZT48bGluZWFyR3JhZGllbnQgaWQ9ImEiIHgxPSIxNzMuMDUiIHkxPSItNjI3Ljc4IiB4Mj0iMTczLjA1IiB5Mj0iLTUyMi40MyIgZ3JhZGllbnRUcmFuc2Zvcm09Im1hdHJpeCgxLjI5LCAwLCAwLCAtMS4zMywgMjcuMTMsIC02MjguMzEpIiBncmFkaWVudFVuaXRzPSJ1c2VyU3BhY2VPblVzZSI+PHN0b3Agb2Zmc2V0PSIwIiBzdG9wLWNvbG9yPSIjZmZmIiBzdG9wLW9wYWNpdHk9IjAuMjUiLz48c3RvcCBvZmZzZXQ9IjEiIHN0b3AtY29sb3I9IiNmZmYiIHN0b3Atb3BhY2l0eT0iMCIvPjwvbGluZWFyR3JhZGllbnQ+PC9kZWZzPjxwYXRoIGNsYXNzPSJhIiBkPSJNNDI5LjMsMTkwLjY2QzQwMi40NSwxMTQuNTEsMzMyLjY3LDYwLjE3LDI1MC44NSw2MC4xN2MtODMuNDMsMC0xNTQuMjgsNTYuNDItMTc5Ljk1LDEzNSwxNS4zNCwzOSw4OC4xMSw3LDE3Ny4wNyw3QzM0MCwyMDIuMDgsNDE3LjI2LDIzNi40Niw0MjkuMywxOTAuNjZaIi8+PC9zdmc+\",\"srcOrientation\":\"Right\"},\"isForeground\":1,\"position\":[0,0,1,1],\"scaleMode\":\"0\"}}],\"derived\":{\"blockParameters\":{\"CustomIcon\":\"data:image\\/svg+xml;base64,PHN2ZyBpZD0iTGF5ZXJfMSIgZGF0YS1uYW1lPSJMYXllciAxIiB4bWxucz0iaHR0cDovL3d3dy53My5vcmcvMjAwMC9zdmciIHZpZXdCb3g9IjAgMCA0MTEgNDU4Ij48ZGVmcz48c3R5bGU+LmNscy0xe2ZpbGw6I2ZkZjhjMTt9LmNscy0ye2ZpbGw6I2ZlZTEwMDt9LmNscy0ze2ZpbGw6IzIzMWYyMDt9LmNscy00e2ZpbGw6I2EwOWY5Zjt9LmNscy00LC5jbHMtNSwuY2xzLTZ7c3Ryb2tlOiMyMzFmMjA7c3Ryb2tlLW1pdGVybGltaXQ6MTA7fS5jbHMtNXtmaWxsOiNmZmY7fS5jbHMtNntmaWxsOm5vbmU7fTwvc3R5bGU+PC9kZWZz ...(+5168 chars)\",\"DefaultColor\":[0.725,0,0],\"Icon\":\"Custom\",\"StateColors\":[{\"color\":[0,0,0],\"value\":\"0\"},{\"color\":[0.4666666666666667,0.6745098039215687,0.18823529411764706],\"value\":\"1\"},{\"color\":[0.5019607843137255,0.5019607843137255,0.5019607843137255],\"value\":\"2\"},{\"color\":[1,0,0],\"value\":\"3\"},{\"color\":[0.07450980392156863,0.6235294117647059,1],\"value\":\"4\"}],\"StateValueType\":\"discrete\",\"fixedAspectRatio\":\"off\"}},\"settings\":{\"BindingType\":\"signal\",\"aspectRatio\":1.032258064516129,\"backgroundColor\":[0,0,0],\"backgroundOffset\":0.14,\"backgroundOpacity\":1,\"blockOrientation\":\"Right\",\"fixedAspectRatio\":\"off\",\"showBackgroundColor\":false,\"value\":0,\"version\":\"R2023a\"},\"type\":\"Lamp\"}"
  RO Mode : CustomWebBlock  LabelPosition=Bottom  ShowInitialText=on  Configuration="{\"components\":[{\"name\":\"BackgroundImageComponent\",\"settings\":{\"image\":{\"size\":[150,150],\"src\":\"data:image\\/svg+xml;base64,PHN2ZyB4bWxucz0iaHR0cDovL3d3dy53My5vcmcvMjAwMC9zdmciIHhtbG5zOnhsaW5rPSJodHRwOi8vd3d3LnczLm9yZy8xOTk5L3hsaW5rIiB2aWV3Qm94PSIwIDAgNTAwIDUwMCI+PGRlZnM+PHN0eWxlPi5he2ZpbGw6dXJsKCNhKTt9LmJ7ZmlsbDp1cmwoI2IpO30uY3tmaWxsOnVybCgjYyk7fTwvc3R5bGU+PHJhZGlhbEdyYWRpZW50IGlkPSJhIiBjeD0iMjgzLjg0IiBjeT0iLTQ2Ni4zNyIgcj0iMzc1Ljc1IiBncmFkaWVudFRyYW5zZm9ybT0ibWF0cml4KDEuMzksIDAsIDAsIC0xLjM5LCAtMTUzLjU2LCAtNjQ0LjA4KSIg ...(+2088 chars)\",\"srcOrientation\":\"Right\"},\"position\":[0,0,1,1],\"scaleMode\":\"0\"}},{\"name\":\"LampStateComponent\",\"settings\":{\"position\":[0,0,1,1],\"states\":[{\"icon\":{\"customSrc\":\"data:image\\/svg+xml;base64,PHN2ZyBpZD0iTGF5ZXJfMSIgZGF0YS1uYW1lPSJMYXllciAxIiB4bWxucz0iaHR0cDovL3d3dy53My5vcmcvMjAwMC9zdmciIHZpZXdCb3g9IjAgMCA0MTEgNDU4Ij48ZGVmcz48c3R5bGU+LmNscy0xe2ZpbGw6I2ZkZjhjMTt9LmNscy0ye2ZpbGw6I2ZlZTEwMDt9LmNscy0ze2ZpbGw6IzIzMWYyMDt9LmNscy00e2ZpbGw6I2EwOWY5Zjt9LmNscy00LC5jbHMtNSwuY2xzLTZ7c3Ryb2tlOiMyMzFmMjA7c3Ryb2tlLW1pdGVybGltaXQ6MTA7fS5jbHMtNXtmaWxsOiNmZmY7fS5jbHMtNntmaWxsOm5vbmU7fTwvc3R5bGU+PC9kZWZz ...(+5168 chars)\",\"id\":-1,\"srcOrientation\":\"Right\",\"type\":\"custom\"},\"iconScale\":0.8,\"metadata\":{},\"overlayType\":\"intersect\",\"shape\":{\"color\":[0.725,0,0],\"opacity\":1,\"position\":[0.1,0.1,0.8,0.8],\"type\":\"ellipse\"},\"value\":[]},{\"icon\":{\"customSrc\":\"data:image\\/svg+xml;base64,PHN2ZyBpZD0iTGF5ZXJfMSIgZGF0YS1uYW1lPSJMYXllciAxIiB4bWxucz0iaHR0cDovL3d3dy53My5vcmcvMjAwMC9zdmciIHZpZXdCb3g9IjAgMCA0MTEgNDU4Ij48ZGVmcz48c3R5bGU+LmNscy0xe2ZpbGw6I2ZkZjhjMTt9LmNscy0ye2ZpbGw6I2ZlZTEwMDt9LmNscy0ze2ZpbGw6IzIzMWYyMDt9LmNscy00e2ZpbGw6I2EwOWY5Zjt9LmNscy00LC5jbHMtNSwuY2xzLTZ7c3Ryb2tlOiMyMzFmMjA7c3Ryb2tlLW1pdGVybGltaXQ6MTA7fS5jbHMtNXtmaWxsOiNmZmY7fS5jbHMtNntmaWxsOm5vbmU7fTwvc3R5bGU+PC9kZWZz ...(+5168 chars)\",\"id\":-1,\"srcOrientation\":\"Right\",\"type\":\"custom\"},\"iconScale\":0.8,\"metadata\":{\"useDefaults\":{\"customIcon\":true,\"icon\":true,\"overlayType\":true,\"shape\":true,\"sizeAndPosition\":true}},\"overlayType\":\"intersect\",\"shape\":{\"color\":[0,0,0],\"opacity\":1,\"position\":[0.1,0.1,0.8,0.8],\"type\":\"ellipse\"},\"value\":\"0\"},{\"icon\":{\"customSrc\":\"data:image\\/svg+xml;base64,PHN2ZyBpZD0iTGF5ZXJfMSIgZGF0YS1uYW1lPSJMYXllciAxIiB4bWxucz0iaHR0cDovL3d3dy53My5vcmcvMjAwMC9zdmciIHZpZXdCb3g9IjAgMCA0MTEgNDU4Ij48ZGVmcz48c3R5bGU+LmNscy0xe2ZpbGw6I2ZkZjhjMTt9LmNscy0ye2ZpbGw6I2ZlZTEwMDt9LmNscy0ze2ZpbGw6IzIzMWYyMDt9LmNscy00e2ZpbGw6I2EwOWY5Zjt9LmNscy00LC5jbHMtNSwuY2xzLTZ7c3Ryb2tlOiMyMzFmMjA7c3Ryb2tlLW1pdGVybGltaXQ6MTA7fS5jbHMtNXtmaWxsOiNmZmY7fS5jbHMtNntmaWxsOm5vbmU7fTwvc3R5bGU+PC9kZWZz ...(+5168 chars)\",\"id\":-1,\"srcOrientation\":\"Right\",\"type\":\"custom\"},\"iconScale\":0.8,\"metadata\":{\"useDefaults\":{\"customIcon\":true,\"icon\":true,\"overlayType\":true,\"shape\":true,\"sizeAndPosition\":true}},\"overlayType\":\"intersect\",\"shape\":{\"color\":[0.4666666666666667,0.6745098039215687,0.18823529411764706],\"opacity\":1,\"position\":[0.1,0.1,0.8,0.8],\"type\":\"ellipse\"},\"value\":\"1\"},{\"icon\":{\"customSrc\":\"data:image\\/svg+xml;base64,PHN2ZyBpZD0iTGF5ZXJfMSIgZGF0YS1uYW1lPSJMYXllciAxIiB4bWxucz0iaHR0cDovL3d3dy53My5vcmcvMjAwMC9zdmciIHZpZXdCb3g9IjAgMCA0MTEgNDU4Ij48ZGVmcz48c3R5bGU+LmNscy0xe2ZpbGw6I2ZkZjhjMTt9LmNscy0ye2ZpbGw6I2ZlZTEwMDt9LmNscy0ze2ZpbGw6IzIzMWYyMDt9LmNscy00e2ZpbGw6I2EwOWY5Zjt9LmNscy00LC5jbHMtNSwuY2xzLTZ7c3Ryb2tlOiMyMzFmMjA7c3Ryb2tlLW1pdGVybGltaXQ6MTA7fS5jbHMtNXtmaWxsOiNmZmY7fS5jbHMtNntmaWxsOm5vbmU7fTwvc3R5bGU+PC9kZWZz ...(+5168 chars)\",\"id\":-1,\"srcOrientation\":\"Right\",\"type\":\"custom\"},\"iconScale\":0.8,\"metadata\":{\"useDefaults\":{\"customIcon\":true,\"icon\":true,\"overlayType\":true,\"shape\":true,\"sizeAndPosition\":true}},\"overlayType\":\"intersect\",\"shape\":{\"color\":[0.5019607843137255,0.5019607843137255,0.5019607843137255],\"opacity\":1,\"position\":[0.1,0.1,0.8,0.8],\"type\":\"ellipse\"},\"value\":\"2\"},{\"icon\":{\"customSrc\":\"data:image\\/svg+xml;base64,PHN2ZyBpZD0iTGF5ZXJfMSIgZGF0YS1uYW1lPSJMYXllciAxIiB4bWxucz0iaHR0cDovL3d3dy53My5vcmcvMjAwMC9zdmciIHZpZXdCb3g9IjAgMCA0MTEgNDU4Ij48ZGVmcz48c3R5bGU+LmNscy0xe2ZpbGw6I2ZkZjhjMTt9LmNscy0ye2ZpbGw6I2ZlZTEwMDt9LmNscy0ze2ZpbGw6IzIzMWYyMDt9LmNscy00e2ZpbGw6I2EwOWY5Zjt9LmNscy00LC5jbHMtNSwuY2xzLTZ7c3Ryb2tlOiMyMzFmMjA7c3Ryb2tlLW1pdGVybGltaXQ6MTA7fS5jbHMtNXtmaWxsOiNmZmY7fS5jbHMtNntmaWxsOm5vbmU7fTwvc3R5bGU+PC9kZWZz ...(+5168 chars)\",\"id\":-1,\"srcOrientation\":\"Right\",\"type\":\"custom\"},\"iconScale\":0.8,\"metadata\":{\"useDefaults\":{\"customIcon\":true,\"icon\":true,\"overlayType\":true,\"shape\":true,\"sizeAndPosition\":true}},\"overlayType\":\"intersect\",\"shape\":{\"color\":[1,0,0],\"opacity\":1,\"position\":[0.1,0.1,0.8,0.8],\"type\":\"ellipse\"},\"value\":\"3\"},{\"icon\":{\"customSrc\":\"data:image\\/svg+xml;base64,PHN2ZyBpZD0iTGF5ZXJfMSIgZGF0YS1uYW1lPSJMYXllciAxIiB4bWxucz0iaHR0cDovL3d3dy53My5vcmcvMjAwMC9zdmciIHZpZXdCb3g9IjAgMCA0MTEgNDU4Ij48ZGVmcz48c3R5bGU+LmNscy0xe2ZpbGw6I2ZkZjhjMTt9LmNscy0ye2ZpbGw6I2ZlZTEwMDt9LmNscy0ze2ZpbGw6IzIzMWYyMDt9LmNscy00e2ZpbGw6I2EwOWY5Zjt9LmNscy00LC5jbHMtNSwuY2xzLTZ7c3Ryb2tlOiMyMzFmMjA7c3Ryb2tlLW1pdGVybGltaXQ6MTA7fS5jbHMtNXtmaWxsOiNmZmY7fS5jbHMtNntmaWxsOm5vbmU7fTwvc3R5bGU+PC9kZWZz ...(+5168 chars)\",\"id\":-1,\"srcOrientation\":\"Right\",\"type\":\"custom\"},\"iconScale\":0.8,\"metadata\":{\"useDefaults\":{\"customIcon\":true,\"icon\":true,\"overlayType\":true,\"shape\":true,\"sizeAndPosition\":true}},\"overlayType\":\"intersect\",\"shape\":{\"color\":[0.07450980392156863,0.6235294117647059,1],\"opacity\":1,\"position\":[0.1,0.1,0.8,0.8],\"type\":\"ellipse\"},\"value\":\"4\"}],\"valueType\":\"discrete\"}},{\"name\":\"ForegroundImageComponent\",\"settings\":{\"image\":{\"size\":[150,150],\"src\":\"data:image\\/svg+xml;base64,PHN2ZyB4bWxucz0iaHR0cDovL3d3dy53My5vcmcvMjAwMC9zdmciIHhtbG5zOnhsaW5rPSJodHRwOi8vd3d3LnczLm9yZy8xOTk5L3hsaW5rIiB2aWV3Qm94PSIwIDAgNTAwIDUwMCI+PGRlZnM+PHN0eWxlPi5he2ZpbGw6dXJsKCNhKTt9PC9zdHlsZT48bGluZWFyR3JhZGllbnQgaWQ9ImEiIHgxPSIxNzMuMDUiIHkxPSItNjI3Ljc4IiB4Mj0iMTczLjA1IiB5Mj0iLTUyMi40MyIgZ3JhZGllbnRUcmFuc2Zvcm09Im1hdHJpeCgxLjI5LCAwLCAwLCAtMS4zMywgMjcuMTMsIC02MjguMzEpIiBncmFkaWVudFVuaXRzPSJ1c2VyU3BhY2VPblVzZSI+PHN0b3Agb2Zmc2V0PSIwIiBzdG9wLWNvbG9yPSIjZmZmIiBzdG9wLW9wYWNpdHk9IjAuMjUiLz48c3RvcCBvZmZzZXQ9IjEiIHN0b3AtY29sb3I9IiNmZmYiIHN0b3Atb3BhY2l0eT0iMCIvPjwvbGluZWFyR3JhZGllbnQ+PC9kZWZzPjxwYXRoIGNsYXNzPSJhIiBkPSJNNDI5LjMsMTkwLjY2QzQwMi40NSwxMTQuNTEsMzMyLjY3LDYwLjE3LDI1MC44NSw2MC4xN2MtODMuNDMsMC0xNTQuMjgsNTYuNDItMTc5Ljk1LDEzNSwxNS4zNCwzOSw4OC4xMSw3LDE3Ny4wNyw3QzM0MCwyMDIuMDgsNDE3LjI2LDIzNi40Niw0MjkuMywxOTAuNjZaIi8+PC9zdmc+\",\"srcOrientation\":\"Right\"},\"isForeground\":1,\"position\":[0,0,1,1],\"scaleMode\":\"0\"}}],\"derived\":{\"blockParameters\":{\"CustomIcon\":\"data:image\\/svg+xml;base64,PHN2ZyBpZD0iTGF5ZXJfMSIgZGF0YS1uYW1lPSJMYXllciAxIiB4bWxucz0iaHR0cDovL3d3dy53My5vcmcvMjAwMC9zdmciIHZpZXdCb3g9IjAgMCA0MTEgNDU4Ij48ZGVmcz48c3R5bGU+LmNscy0xe2ZpbGw6I2ZkZjhjMTt9LmNscy0ye2ZpbGw6I2ZlZTEwMDt9LmNscy0ze2ZpbGw6IzIzMWYyMDt9LmNscy00e2ZpbGw6I2EwOWY5Zjt9LmNscy00LC5jbHMtNSwuY2xzLTZ7c3Ryb2tlOiMyMzFmMjA7c3Ryb2tlLW1pdGVybGltaXQ6MTA7fS5jbHMtNXtmaWxsOiNmZmY7fS5jbHMtNntmaWxsOm5vbmU7fTwvc3R5bGU+PC9kZWZz ...(+5168 chars)\",\"DefaultColor\":[0.725,0,0],\"Icon\":\"Custom\",\"StateColors\":[{\"color\":[0,0,0],\"value\":\"0\"},{\"color\":[0.4666666666666667,0.6745098039215687,0.18823529411764706],\"value\":\"1\"},{\"color\":[0.5019607843137255,0.5019607843137255,0.5019607843137255],\"value\":\"2\"},{\"color\":[1,0,0],\"value\":\"3\"},{\"color\":[0.07450980392156863,0.6235294117647059,1],\"value\":\"4\"}],\"StateValueType\":\"discrete\",\"fixedAspectRatio\":\"off\"}},\"settings\":{\"BindingType\":\"signal\",\"aspectRatio\":1.032258064516129,\"backgroundColor\":[0,0,0],\"backgroundOffset\":0.14,\"backgroundOpacity\":1,\"blockOrientation\":\"Right\",\"fixedAspectRatio\":\"off\",\"showBackgroundColor\":false,\"value\":0,\"version\":\"R2023a\"},\"type\":\"Lamp\"}"
  Remote Electronic Units : Subsystem  TreatAsAtomicUnit=on  SystemSampleTime=.01
      settings: PortSchema="{\"entries\":[{\"content\":{\"sides\":[{\"content\":{\"connectorIds\":[\"In1\",\"Out2\"]},\"type\":\"ConnectorPlacement.EquallySpacedRectSide\",\"uuid\":\"38682bff-efe9-4f74-b563-7d17327409bc\"},{\"content\":{\"connectorIds\":[\"Out1\",\"In2\"],\"side\":\"RIGHT\"},\"type\":\"ConnectorPlacement.EquallySpacedRectSide\",\"uuid\":\"9b27296a-7a15-43c2-9a49-3690713ba5ee\"},{\"content\":{\"side\":\"TOP\"},\"type\":\"ConnectorPlacement.EquallySpacedRectSide\",\"uuid\":\"df0d1eaf-2d63-4586-9b70-ab9eb3cbba48\"}]},\"type\":\"ConnectorPlacement.EquallySpacedConnector\",\"uuid\":\"3720bb81-e23a-4071-aa80-868b0be59702\"}],\"packageUris\":[\"http://schema.mathworks.com/mf0/Connector/R2020b\"],\"version\":\"1.0\"}"
  Slider Switch : CustomTuningWebBlock  LabelPosition=Hide  ShowInitialText=on  Configuration="{\"components\":[{\"name\":\"CustomSwitchStateComponent\",\"settings\":{\"position\":[0,0,1,1],\"states\":[{\"HitRegion\":{\"position\":[0,0,0.5,1]},\"Image\":{\"position\":[0,0,1,1],\"size\":[1,1],\"src\":\"data:image\\/svg+xml;base64,PD94bWwgdmVyc2lvbj0iMS4wIiBlbmNvZGluZz0idXRmLTgiPz4NCjwhLS0gR2VuZXJhdG9yOiBBZG9iZSBJbGx1c3RyYXRvciAyNS4yLjEsIFNWRyBFeHBvcnQgUGx1Zy1JbiAuIFNWRyBWZXJzaW9uOiA2LjAwIEJ1aWxkIDApICAtLT4NCjxzdmcgdmVyc2lvbj0iMS4xIiB4bWxucz0iaHR0cDovL3d3dy53My5vcmcvMjAwMC9zdmciIHhtbG5zOnhsaW5rPSJodHRwOi8vd3d3LnczLm9yZy8xOTk5L3hsaW5rIiB4PSIwcHgiIHk9IjBweCINCgkgdmlld0JveD0iMCAwIDc2IDI5IiBzdHlsZT0iZW5hYmxlLWJhY2tncm91bmQ6bmV3 ...(+5404 chars)\",\"srcOrientation\":\"Right\"},\"Label\":{\"color\":[0.9882352941176471,0.9882352941176471,0.7725490196078432],\"icon\":{\"size\":[0,0],\"src\":[],\"srcOrientation\":\"Right\"},\"iconOffset\":0,\"iconPlacement\":\"left\",\"opacity\":1,\"position\":[0.5,0.14],\"show\":true,\"text\":{\"content\":\"LO\",\"font\":\"Helvetica\"}},\"Value\":0},{\"HitRegion\":{\"position\":[0,0.5,0.5,1]},\"Image\":{\"position\":[0,0,1,1],\"size\":[1,1],\"src\":\"data:image\\/svg+xml;base64,PD94bWwgdmVyc2lvbj0iMS4wIiBlbmNvZGluZz0idXRmLTgiPz4NCjwhLS0gR2VuZXJhdG9yOiBBZG9iZSBJbGx1c3RyYXRvciAyNS4yLjEsIFNWRyBFeHBvcnQgUGx1Zy1JbiAuIFNWRyBWZXJzaW9uOiA2LjAwIEJ1aWxkIDApICAtLT4NCjxzdmcgdmVyc2lvbj0iMS4xIiB4bWxucz0iaHR0cDovL3d3dy53My5vcmcvMjAwMC9zdmciIHhtbG5zOnhsaW5rPSJodHRwOi8vd3d3LnczLm9yZy8xOTk5L3hsaW5rIiB4PSIwcHgiIHk9IjBweCINCgkgdmlld0JveD0iMCAwIDc2IDI5IiBzdHlsZT0iZW5hYmxlLWJhY2tncm91bmQ6bmV3 ...(+5404 chars)\",\"srcOrientation\":\"Right\"},\"Label\":{\"color\":[0.9882352941176471,0.9882352941176471,0.7725490196078432],\"icon\":{\"size\":[0,0],\"src\":[],\"srcOrientation\":\"Right\"},\"iconOffset\":0,\"iconPlacement\":\"left\",\"opacity\":1,\"position\":[0.5,0.86],\"show\":true,\"text\":{\"content\":\"\",\"font\":\"Helvetica\"}},\"Value\":1}]}},{\"name\":\"BackgroundImageComponent\",\"settings\":{\"image\":{\"size\":[140,55],\"src\":\"default\",\"srcOrientation\":\"Right\"},\"position\":[0,0,1,1],\"scaleMode\":\"0\"}},{\"name\":\"ForegroundImageComponent\",\"settings\":{\"image\":{\"size\":[0,0],\"src\":\"default\",\"srcOrientation\":[]},\"isForeground\":1,\"position\":[0,0,1,1],\"scaleMode\":\"0\"}}],\"derived\":{\"blockParameters\":{\"StatesJSON\":[{\"Label\":\"LO\",\"Value\":0},{\"Label\":\"\",\"Value\":1}],\"fixedAspectRatio\":\"on\"}},\"settings\":{\"BindingType\":\"param\",\"backgroundColor\":[0,0,255,\"1\"],\"backgroundOffset\":0.14,\"fixedAspectRatio\":\"on\",\"foregroundColor\":[234,234,234],\"showBackgroundColor\":false,\"variant\":\"slider\",\"version\":\"R2024b\"},\"type\":\"Switch\"}"
  Slider Switch1 : CustomTuningWebBlock  LabelPosition=Hide  ShowInitialText=on  Configuration="{\"components\":[{\"name\":\"CustomSwitchStateComponent\",\"settings\":{\"position\":[0,0,1,1],\"states\":[{\"HitRegion\":{\"position\":[0,0,0.5,1]},\"Image\":{\"position\":[0,0,1,1],\"size\":[1,1],\"src\":\"data:image\\/svg+xml;base64,PD94bWwgdmVyc2lvbj0iMS4wIiBlbmNvZGluZz0idXRmLTgiPz4NCjwhLS0gR2VuZXJhdG9yOiBBZG9iZSBJbGx1c3RyYXRvciAyNS4yLjEsIFNWRyBFeHBvcnQgUGx1Zy1JbiAuIFNWRyBWZXJzaW9uOiA2LjAwIEJ1aWxkIDApICAtLT4NCjxzdmcgdmVyc2lvbj0iMS4xIiB4bWxucz0iaHR0cDovL3d3dy53My5vcmcvMjAwMC9zdmciIHhtbG5zOnhsaW5rPSJodHRwOi8vd3d3LnczLm9yZy8xOTk5L3hsaW5rIiB4PSIwcHgiIHk9IjBweCINCgkgdmlld0JveD0iMCAwIDc2IDI5IiBzdHlsZT0iZW5hYmxlLWJhY2tncm91bmQ6bmV3 ...(+5404 chars)\",\"srcOrientation\":\"Right\"},\"Label\":{\"color\":[0.9882352941176471,0.9882352941176471,0.7725490196078432],\"icon\":{\"size\":[0,0],\"src\":[],\"srcOrientation\":\"Right\"},\"iconOffset\":0,\"iconPlacement\":\"left\",\"opacity\":1,\"position\":[0.5,0.14],\"show\":true,\"text\":{\"content\":\"LI\",\"font\":\"Helvetica\"}},\"Value\":0},{\"HitRegion\":{\"position\":[0,0.5,0.5,1]},\"Image\":{\"position\":[0,0,1,1],\"size\":[1,1],\"src\":\"data:image\\/svg+xml;base64,PD94bWwgdmVyc2lvbj0iMS4wIiBlbmNvZGluZz0idXRmLTgiPz4NCjwhLS0gR2VuZXJhdG9yOiBBZG9iZSBJbGx1c3RyYXRvciAyNS4yLjEsIFNWRyBFeHBvcnQgUGx1Zy1JbiAuIFNWRyBWZXJzaW9uOiA2LjAwIEJ1aWxkIDApICAtLT4NCjxzdmcgdmVyc2lvbj0iMS4xIiB4bWxucz0iaHR0cDovL3d3dy53My5vcmcvMjAwMC9zdmciIHhtbG5zOnhsaW5rPSJodHRwOi8vd3d3LnczLm9yZy8xOTk5L3hsaW5rIiB4PSIwcHgiIHk9IjBweCINCgkgdmlld0JveD0iMCAwIDc2IDI5IiBzdHlsZT0iZW5hYmxlLWJhY2tncm91bmQ6bmV3 ...(+5404 chars)\",\"srcOrientation\":\"Right\"},\"Label\":{\"color\":[0.9882352941176471,0.9882352941176471,0.7725490196078432],\"icon\":{\"size\":[0,0],\"src\":[],\"srcOrientation\":\"Right\"},\"iconOffset\":0,\"iconPlacement\":\"left\",\"opacity\":1,\"position\":[0.5,0.86],\"show\":true,\"text\":{\"content\":\"\",\"font\":\"Helvetica\"}},\"Value\":1}]}},{\"name\":\"BackgroundImageComponent\",\"settings\":{\"image\":{\"size\":[140,55],\"src\":\"default\",\"srcOrientation\":\"Right\"},\"position\":[0,0,1,1],\"scaleMode\":\"0\"}},{\"name\":\"ForegroundImageComponent\",\"settings\":{\"image\":{\"size\":[0,0],\"src\":\"default\",\"srcOrientation\":[]},\"isForeground\":1,\"position\":[0,0,1,1],\"scaleMode\":\"0\"}}],\"derived\":{\"blockParameters\":{\"StatesJSON\":[{\"Label\":\"LI\",\"Value\":0},{\"Label\":\"\",\"Value\":1}],\"fixedAspectRatio\":\"on\"}},\"settings\":{\"BindingType\":\"param\",\"backgroundColor\":[0,0,255,\"1\"],\"backgroundOffset\":0.14,\"fixedAspectRatio\":\"on\",\"foregroundColor\":[234,234,234],\"showBackgroundColor\":false,\"variant\":\"slider\",\"version\":\"R2024b\"},\"type\":\"Switch\"}"
  Slider Switch2 : CustomTuningWebBlock  LabelPosition=Hide  ShowInitialText=on  Configuration="{\"components\":[{\"name\":\"CustomSwitchStateComponent\",\"settings\":{\"position\":[0,0,1,1],\"states\":[{\"HitRegion\":{\"position\":[0,0,0.5,1]},\"Image\":{\"position\":[0,0,1,1],\"size\":[1,1],\"src\":\"data:image\\/svg+xml;base64,PD94bWwgdmVyc2lvbj0iMS4wIiBlbmNvZGluZz0idXRmLTgiPz4NCjwhLS0gR2VuZXJhdG9yOiBBZG9iZSBJbGx1c3RyYXRvciAyNS4yLjEsIFNWRyBFeHBvcnQgUGx1Zy1JbiAuIFNWRyBWZXJzaW9uOiA2LjAwIEJ1aWxkIDApICAtLT4NCjxzdmcgdmVyc2lvbj0iMS4xIiB4bWxucz0iaHR0cDovL3d3dy53My5vcmcvMjAwMC9zdmciIHhtbG5zOnhsaW5rPSJodHRwOi8vd3d3LnczLm9yZy8xOTk5L3hsaW5rIiB4PSIwcHgiIHk9IjBweCINCgkgdmlld0JveD0iMCAwIDc2IDI5IiBzdHlsZT0iZW5hYmxlLWJhY2tncm91bmQ6bmV3 ...(+5404 chars)\",\"srcOrientation\":\"Right\"},\"Label\":{\"color\":[0.9882352941176471,0.9882352941176471,0.7725490196078432],\"icon\":{\"size\":[0,0],\"src\":[],\"srcOrientation\":\"Right\"},\"iconOffset\":0,\"iconPlacement\":\"left\",\"opacity\":1,\"position\":[0.5,0.14],\"show\":true,\"text\":{\"content\":\"RI\",\"font\":\"Helvetica\"}},\"Value\":0},{\"HitRegion\":{\"position\":[0,0.5,0.5,1]},\"Image\":{\"position\":[0,0,1,1],\"size\":[1,1],\"src\":\"data:image\\/svg+xml;base64,PD94bWwgdmVyc2lvbj0iMS4wIiBlbmNvZGluZz0idXRmLTgiPz4NCjwhLS0gR2VuZXJhdG9yOiBBZG9iZSBJbGx1c3RyYXRvciAyNS4yLjEsIFNWRyBFeHBvcnQgUGx1Zy1JbiAuIFNWRyBWZXJzaW9uOiA2LjAwIEJ1aWxkIDApICAtLT4NCjxzdmcgdmVyc2lvbj0iMS4xIiB4bWxucz0iaHR0cDovL3d3dy53My5vcmcvMjAwMC9zdmciIHhtbG5zOnhsaW5rPSJodHRwOi8vd3d3LnczLm9yZy8xOTk5L3hsaW5rIiB4PSIwcHgiIHk9IjBweCINCgkgdmlld0JveD0iMCAwIDc2IDI5IiBzdHlsZT0iZW5hYmxlLWJhY2tncm91bmQ6bmV3 ...(+5404 chars)\",\"srcOrientation\":\"Right\"},\"Label\":{\"color\":[0.9882352941176471,0.9882352941176471,0.7725490196078432],\"icon\":{\"size\":[0,0],\"src\":[],\"srcOrientation\":\"Right\"},\"iconOffset\":0,\"iconPlacement\":\"left\",\"opacity\":1,\"position\":[0.5,0.86],\"show\":true,\"text\":{\"content\":\"\",\"font\":\"Helvetica\"}},\"Value\":1}]}},{\"name\":\"BackgroundImageComponent\",\"settings\":{\"image\":{\"size\":[140,55],\"src\":\"default\",\"srcOrientation\":\"Right\"},\"position\":[0,0,1,1],\"scaleMode\":\"0\"}},{\"name\":\"ForegroundImageComponent\",\"settings\":{\"image\":{\"size\":[0,0],\"src\":\"default\",\"srcOrientation\":[]},\"isForeground\":1,\"position\":[0,0,1,1],\"scaleMode\":\"0\"}}],\"derived\":{\"blockParameters\":{\"StatesJSON\":[{\"Label\":\"RI\",\"Value\":0},{\"Label\":\"\",\"Value\":1}],\"fixedAspectRatio\":\"on\"}},\"settings\":{\"BindingType\":\"param\",\"backgroundColor\":[0,0,255,\"1\"],\"backgroundOffset\":0.14,\"fixedAspectRatio\":\"on\",\"foregroundColor\":[234,234,234],\"showBackgroundColor\":false,\"variant\":\"slider\",\"version\":\"R2024b\"},\"type\":\"Switch\"}"
  Slider Switch3 : CustomTuningWebBlock  LabelPosition=Hide  ShowInitialText=on  Configuration="{\"components\":[{\"name\":\"CustomSwitchStateComponent\",\"settings\":{\"position\":[0,0,1,1],\"states\":[{\"HitRegion\":{\"position\":[0,0,0.5,1]},\"Image\":{\"position\":[0,0,1,1],\"size\":[1,1],\"src\":\"data:image\\/svg+xml;base64,PD94bWwgdmVyc2lvbj0iMS4wIiBlbmNvZGluZz0idXRmLTgiPz4NCjwhLS0gR2VuZXJhdG9yOiBBZG9iZSBJbGx1c3RyYXRvciAyNS4yLjEsIFNWRyBFeHBvcnQgUGx1Zy1JbiAuIFNWRyBWZXJzaW9uOiA2LjAwIEJ1aWxkIDApICAtLT4NCjxzdmcgdmVyc2lvbj0iMS4xIiB4bWxucz0iaHR0cDovL3d3dy53My5vcmcvMjAwMC9zdmciIHhtbG5zOnhsaW5rPSJodHRwOi8vd3d3LnczLm9yZy8xOTk5L3hsaW5rIiB4PSIwcHgiIHk9IjBweCINCgkgdmlld0JveD0iMCAwIDc2IDI5IiBzdHlsZT0iZW5hYmxlLWJhY2tncm91bmQ6bmV3 ...(+5404 chars)\",\"srcOrientation\":\"Right\"},\"Label\":{\"color\":[0.9882352941176471,0.9882352941176471,0.7725490196078432],\"icon\":{\"size\":[0,0],\"src\":[],\"srcOrientation\":\"Right\"},\"iconOffset\":0,\"iconPlacement\":\"left\",\"opacity\":1,\"position\":[0.5,0.14],\"show\":true,\"text\":{\"content\":\"RO\",\"font\":\"Helvetica\"}},\"Value\":0},{\"HitRegion\":{\"position\":[0,0.5,0.5,1]},\"Image\":{\"position\":[0,0,1,1],\"size\":[1,1],\"src\":\"data:image\\/svg+xml;base64,PD94bWwgdmVyc2lvbj0iMS4wIiBlbmNvZGluZz0idXRmLTgiPz4NCjwhLS0gR2VuZXJhdG9yOiBBZG9iZSBJbGx1c3RyYXRvciAyNS4yLjEsIFNWRyBFeHBvcnQgUGx1Zy1JbiAuIFNWRyBWZXJzaW9uOiA2LjAwIEJ1aWxkIDApICAtLT4NCjxzdmcgdmVyc2lvbj0iMS4xIiB4bWxucz0iaHR0cDovL3d3dy53My5vcmcvMjAwMC9zdmciIHhtbG5zOnhsaW5rPSJodHRwOi8vd3d3LnczLm9yZy8xOTk5L3hsaW5rIiB4PSIwcHgiIHk9IjBweCINCgkgdmlld0JveD0iMCAwIDc2IDI5IiBzdHlsZT0iZW5hYmxlLWJhY2tncm91bmQ6bmV3 ...(+5404 chars)\",\"srcOrientation\":\"Right\"},\"Label\":{\"color\":[0.9882352941176471,0.9882352941176471,0.7725490196078432],\"icon\":{\"size\":[0,0],\"src\":[],\"srcOrientation\":\"Right\"},\"iconOffset\":0,\"iconPlacement\":\"left\",\"opacity\":1,\"position\":[0.5,0.86],\"show\":true,\"text\":{\"content\":\"\",\"font\":\"Helvetica\"}},\"Value\":1}]}},{\"name\":\"BackgroundImageComponent\",\"settings\":{\"image\":{\"size\":[140,55],\"src\":\"default\",\"srcOrientation\":\"Right\"},\"position\":[0,0,1,1],\"scaleMode\":\"0\"}},{\"name\":\"ForegroundImageComponent\",\"settings\":{\"image\":{\"size\":[0,0],\"src\":\"default\",\"srcOrientation\":[]},\"isForeground\":1,\"position\":[0,0,1,1],\"scaleMode\":\"0\"}}],\"derived\":{\"blockParameters\":{\"StatesJSON\":[{\"Label\":\"RO\",\"Value\":0},{\"Label\":\"\",\"Value\":1}],\"fixedAspectRatio\":\"on\"}},\"settings\":{\"BindingType\":\"param\",\"backgroundColor\":[0,0,255,\"1\"],\"backgroundOffset\":0.14,\"fixedAspectRatio\":\"on\",\"foregroundColor\":[234,234,234],\"showBackgroundColor\":false,\"variant\":\"slider\",\"version\":\"R2024b\"},\"type\":\"Switch\"}"
  Slider Switch4 : CustomTuningWebBlock  LabelPosition=Hide  ShowInitialText=on  Configuration="{\"components\":[{\"name\":\"CustomSwitchStateComponent\",\"settings\":{\"position\":[0,0,1,1],\"states\":[{\"HitRegion\":{\"position\":[0,0,0.5,1]},\"Image\":{\"position\":[0,0,1,1],\"size\":[1,1],\"src\":\"data:image\\/svg+xml;base64,PD94bWwgdmVyc2lvbj0iMS4wIiBlbmNvZGluZz0idXRmLTgiPz4NCjwhLS0gR2VuZXJhdG9yOiBBZG9iZSBJbGx1c3RyYXRvciAyNS4yLjEsIFNWRyBFeHBvcnQgUGx1Zy1JbiAuIFNWRyBWZXJzaW9uOiA2LjAwIEJ1aWxkIDApICAtLT4NCjxzdmcgdmVyc2lvbj0iMS4xIiB4bWxucz0iaHR0cDovL3d3dy53My5vcmcvMjAwMC9zdmciIHhtbG5zOnhsaW5rPSJodHRwOi8vd3d3LnczLm9yZy8xOTk5L3hsaW5rIiB4PSIwcHgiIHk9IjBweCINCgkgdmlld0JveD0iMCAwIDc2IDI5IiBzdHlsZT0iZW5hYmxlLWJhY2tncm91bmQ6bmV3 ...(+5404 chars)\",\"srcOrientation\":\"Right\"},\"Label\":{\"color\":[0.9882352941176471,0.9882352941176471,0.7725490196078432],\"icon\":{\"size\":[0,0],\"src\":[],\"srcOrientation\":\"Right\"},\"iconOffset\":0,\"iconPlacement\":\"left\",\"opacity\":1,\"position\":[0.5,0.14],\"show\":true,\"text\":{\"content\":\"H1\",\"font\":\"Helvetica\"}},\"Value\":0},{\"HitRegion\":{\"position\":[0,0.5,0.5,1]},\"Image\":{\"position\":[0,0,1,1],\"size\":[1,1],\"src\":\"data:image\\/svg+xml;base64,PD94bWwgdmVyc2lvbj0iMS4wIiBlbmNvZGluZz0idXRmLTgiPz4NCjwhLS0gR2VuZXJhdG9yOiBBZG9iZSBJbGx1c3RyYXRvciAyNS4yLjEsIFNWRyBFeHBvcnQgUGx1Zy1JbiAuIFNWRyBWZXJzaW9uOiA2LjAwIEJ1aWxkIDApICAtLT4NCjxzdmcgdmVyc2lvbj0iMS4xIiB4bWxucz0iaHR0cDovL3d3dy53My5vcmcvMjAwMC9zdmciIHhtbG5zOnhsaW5rPSJodHRwOi8vd3d3LnczLm9yZy8xOTk5L3hsaW5rIiB4PSIwcHgiIHk9IjBweCINCgkgdmlld0JveD0iMCAwIDc2IDI5IiBzdHlsZT0iZW5hYmxlLWJhY2tncm91bmQ6bmV3 ...(+5404 chars)\",\"srcOrientation\":\"Right\"},\"Label\":{\"color\":[0.9882352941176471,0.9882352941176471,0.7725490196078432],\"icon\":{\"size\":[0,0],\"src\":[],\"srcOrientation\":\"Right\"},\"iconOffset\":0,\"iconPlacement\":\"left\",\"opacity\":1,\"position\":[0.5,0.86],\"show\":true,\"text\":{\"content\":\"\",\"font\":\"Helvetica\"}},\"Value\":1}]}},{\"name\":\"BackgroundImageComponent\",\"settings\":{\"image\":{\"size\":[140,55],\"src\":\"default\",\"srcOrientation\":\"Right\"},\"position\":[0,0,1,1],\"scaleMode\":\"0\"}},{\"name\":\"ForegroundImageComponent\",\"settings\":{\"image\":{\"size\":[0,0],\"src\":\"default\",\"srcOrientation\":[]},\"isForeground\":1,\"position\":[0,0,1,1],\"scaleMode\":\"0\"}}],\"derived\":{\"blockParameters\":{\"StatesJSON\":[{\"Label\":\"H1\",\"Value\":0},{\"Label\":\"\",\"Value\":1}],\"fixedAspectRatio\":\"on\"}},\"settings\":{\"BindingType\":\"param\",\"backgroundColor\":[0,0,255,\"1\"],\"backgroundOffset\":0.14,\"fixedAspectRatio\":\"on\",\"foregroundColor\":[234,234,234],\"showBackgroundColor\":false,\"variant\":\"slider\",\"version\":\"R2024b\"},\"type\":\"Switch\"}"
  Slider Switch5 : CustomTuningWebBlock  LabelPosition=Hide  ShowInitialText=on  Configuration="{\"components\":[{\"name\":\"CustomSwitchStateComponent\",\"settings\":{\"position\":[0,0,1,1],\"states\":[{\"HitRegion\":{\"position\":[0,0,0.5,1]},\"Image\":{\"position\":[0,0,1,1],\"size\":[1,1],\"src\":\"data:image\\/svg+xml;base64,PD94bWwgdmVyc2lvbj0iMS4wIiBlbmNvZGluZz0idXRmLTgiPz4NCjwhLS0gR2VuZXJhdG9yOiBBZG9iZSBJbGx1c3RyYXRvciAyNS4yLjEsIFNWRyBFeHBvcnQgUGx1Zy1JbiAuIFNWRyBWZXJzaW9uOiA2LjAwIEJ1aWxkIDApICAtLT4NCjxzdmcgdmVyc2lvbj0iMS4xIiB4bWxucz0iaHR0cDovL3d3dy53My5vcmcvMjAwMC9zdmciIHhtbG5zOnhsaW5rPSJodHRwOi8vd3d3LnczLm9yZy8xOTk5L3hsaW5rIiB4PSIwcHgiIHk9IjBweCINCgkgdmlld0JveD0iMCAwIDc2IDI5IiBzdHlsZT0iZW5hYmxlLWJhY2tncm91bmQ6bmV3 ...(+5404 chars)\",\"srcOrientation\":\"Right\"},\"Label\":{\"color\":[0.9882352941176471,0.9882352941176471,0.7725490196078432],\"icon\":{\"size\":[0,0],\"src\":[],\"srcOrientation\":\"Right\"},\"iconOffset\":0,\"iconPlacement\":\"left\",\"opacity\":1,\"position\":[0.5,0.14],\"show\":true,\"text\":{\"content\":\"H2\",\"font\":\"Helvetica\"}},\"Value\":0},{\"HitRegion\":{\"position\":[0,0.5,0.5,1]},\"Image\":{\"position\":[0,0,1,1],\"size\":[1,1],\"src\":\"data:image\\/svg+xml;base64,PD94bWwgdmVyc2lvbj0iMS4wIiBlbmNvZGluZz0idXRmLTgiPz4NCjwhLS0gR2VuZXJhdG9yOiBBZG9iZSBJbGx1c3RyYXRvciAyNS4yLjEsIFNWRyBFeHBvcnQgUGx1Zy1JbiAuIFNWRyBWZXJzaW9uOiA2LjAwIEJ1aWxkIDApICAtLT4NCjxzdmcgdmVyc2lvbj0iMS4xIiB4bWxucz0iaHR0cDovL3d3dy53My5vcmcvMjAwMC9zdmciIHhtbG5zOnhsaW5rPSJodHRwOi8vd3d3LnczLm9yZy8xOTk5L3hsaW5rIiB4PSIwcHgiIHk9IjBweCINCgkgdmlld0JveD0iMCAwIDc2IDI5IiBzdHlsZT0iZW5hYmxlLWJhY2tncm91bmQ6bmV3 ...(+5404 chars)\",\"srcOrientation\":\"Right\"},\"Label\":{\"color\":[0.9882352941176471,0.9882352941176471,0.7725490196078432],\"icon\":{\"size\":[0,0],\"src\":[],\"srcOrientation\":\"Right\"},\"iconOffset\":0,\"iconPlacement\":\"left\",\"opacity\":1,\"position\":[0.5,0.86],\"show\":true,\"text\":{\"content\":\"\",\"font\":\"Helvetica\"}},\"Value\":1}]}},{\"name\":\"BackgroundImageComponent\",\"settings\":{\"image\":{\"size\":[140,55],\"src\":\"default\",\"srcOrientation\":\"Right\"},\"position\":[0,0,1,1],\"scaleMode\":\"0\"}},{\"name\":\"ForegroundImageComponent\",\"settings\":{\"image\":{\"size\":[0,0],\"src\":\"default\",\"srcOrientation\":[]},\"isForeground\":1,\"position\":[0,0,1,1],\"scaleMode\":\"0\"}}],\"derived\":{\"blockParameters\":{\"StatesJSON\":[{\"Label\":\"H2\",\"Value\":0},{\"Label\":\"\",\"Value\":1}],\"fixedAspectRatio\":\"on\"}},\"settings\":{\"BindingType\":\"param\",\"backgroundColor\":[0,0,255,\"1\"],\"backgroundOffset\":0.14,\"fixedAspectRatio\":\"on\",\"foregroundColor\":[234,234,234],\"showBackgroundColor\":false,\"variant\":\"slider\",\"version\":\"R2024b\"},\"type\":\"Switch\"}"
  Slider Switch6 : CustomTuningWebBlock  LabelPosition=Hide  ShowInitialText=on  Configuration="{\"components\":[{\"name\":\"CustomSwitchStateComponent\",\"settings\":{\"position\":[0,0,1,1],\"states\":[{\"HitRegion\":{\"position\":[0,0,0.5,1]},\"Image\":{\"position\":[0,0,1,1],\"size\":[1,1],\"src\":\"data:image\\/svg+xml;base64,PD94bWwgdmVyc2lvbj0iMS4wIiBlbmNvZGluZz0idXRmLTgiPz4NCjwhLS0gR2VuZXJhdG9yOiBBZG9iZSBJbGx1c3RyYXRvciAyNS4yLjEsIFNWRyBFeHBvcnQgUGx1Zy1JbiAuIFNWRyBWZXJzaW9uOiA2LjAwIEJ1aWxkIDApICAtLT4NCjxzdmcgdmVyc2lvbj0iMS4xIiB4bWxucz0iaHR0cDovL3d3dy53My5vcmcvMjAwMC9zdmciIHhtbG5zOnhsaW5rPSJodHRwOi8vd3d3LnczLm9yZy8xOTk5L3hsaW5rIiB4PSIwcHgiIHk9IjBweCINCgkgdmlld0JveD0iMCAwIDc2IDI5IiBzdHlsZT0iZW5hYmxlLWJhY2tncm91bmQ6bmV3 ...(+5404 chars)\",\"srcOrientation\":\"Right\"},\"Label\":{\"color\":[0.9882352941176471,0.9882352941176471,0.7725490196078432],\"icon\":{\"size\":[0,0],\"src\":[],\"srcOrientation\":\"Right\"},\"iconOffset\":0,\"iconPlacement\":\"left\",\"opacity\":1,\"position\":[0.5,0.14],\"show\":true,\"text\":{\"content\":\"H3\",\"font\":\"Helvetica\"}},\"Value\":0},{\"HitRegion\":{\"position\":[0,0.5,0.5,1]},\"Image\":{\"position\":[0,0,1,1],\"size\":[1,1],\"src\":\"data:image\\/svg+xml;base64,PD94bWwgdmVyc2lvbj0iMS4wIiBlbmNvZGluZz0idXRmLTgiPz4NCjwhLS0gR2VuZXJhdG9yOiBBZG9iZSBJbGx1c3RyYXRvciAyNS4yLjEsIFNWRyBFeHBvcnQgUGx1Zy1JbiAuIFNWRyBWZXJzaW9uOiA2LjAwIEJ1aWxkIDApICAtLT4NCjxzdmcgdmVyc2lvbj0iMS4xIiB4bWxucz0iaHR0cDovL3d3dy53My5vcmcvMjAwMC9zdmciIHhtbG5zOnhsaW5rPSJodHRwOi8vd3d3LnczLm9yZy8xOTk5L3hsaW5rIiB4PSIwcHgiIHk9IjBweCINCgkgdmlld0JveD0iMCAwIDc2IDI5IiBzdHlsZT0iZW5hYmxlLWJhY2tncm91bmQ6bmV3 ...(+5404 chars)\",\"srcOrientation\":\"Right\"},\"Label\":{\"color\":[0.9882352941176471,0.9882352941176471,0.7725490196078432],\"icon\":{\"size\":[0,0],\"src\":[],\"srcOrientation\":\"Right\"},\"iconOffset\":0,\"iconPlacement\":\"left\",\"opacity\":1,\"position\":[0.5,0.86],\"show\":true,\"text\":{\"content\":\"\",\"font\":\"Helvetica\"}},\"Value\":1}]}},{\"name\":\"BackgroundImageComponent\",\"settings\":{\"image\":{\"size\":[140,55],\"src\":\"default\",\"srcOrientation\":\"Right\"},\"position\":[0,0,1,1],\"scaleMode\":\"0\"}},{\"name\":\"ForegroundImageComponent\",\"settings\":{\"image\":{\"size\":[0,0],\"src\":\"default\",\"srcOrientation\":[]},\"isForeground\":1,\"position\":[0,0,1,1],\"scaleMode\":\"0\"}}],\"derived\":{\"blockParameters\":{\"StatesJSON\":[{\"Label\":\"H3\",\"Value\":0},{\"Label\":\"\",\"Value\":1}],\"fixedAspectRatio\":\"on\"}},\"settings\":{\"BindingType\":\"param\",\"backgroundColor\":[0,0,255,\"1\"],\"backgroundOffset\":0.14,\"fixedAspectRatio\":\"on\",\"foregroundColor\":[234,234,234],\"showBackgroundColor\":false,\"variant\":\"slider\",\"version\":\"R2024b\"},\"type\":\"Switch\"}"
  Scope : Scope
      settings: ActiveDisplayYMinimum=-1.38385  ActiveDisplayYMaximum=1.37745
  modes : Scope
      settings: TimeSpan=20  ActiveDisplayYMinimum=0  ActiveDisplayYMaximum=4.5  DataLoggingMaxPoints=7500  DataLoggingSaveFormat=Array
  wires:
  Pilot/1 -> Primary Flight Control Computer/1  "PilotCmd"
  Primary Flight Control Computer/1 -> Remote Electronic Units/1(To REUs)
  Remote Electronic Units/1(To Plant) -> Plant/1(To Plant)
  Plant/1(FromPlant) -> Remote Electronic Units/2(From Plant)
  Remote Electronic Units/2(From REUs) -> Primary Flight Control Computer/2
